simulink model "solar_pv_protected_c07_circuit"  (R2026b)
settings: Solver=VariableStepAuto
model workspace (MAT data in the model file):
  candidate_owner = 'pv_protection_integration_20261023_r01'
  solar_edit_metadata : object (value not decoded)
libraries: fl_lib x149, ee_lib x16, ltc4364demo_lib x3, batteryecm_lib x1, solarprotect_lib x1
(part 11 of 16)

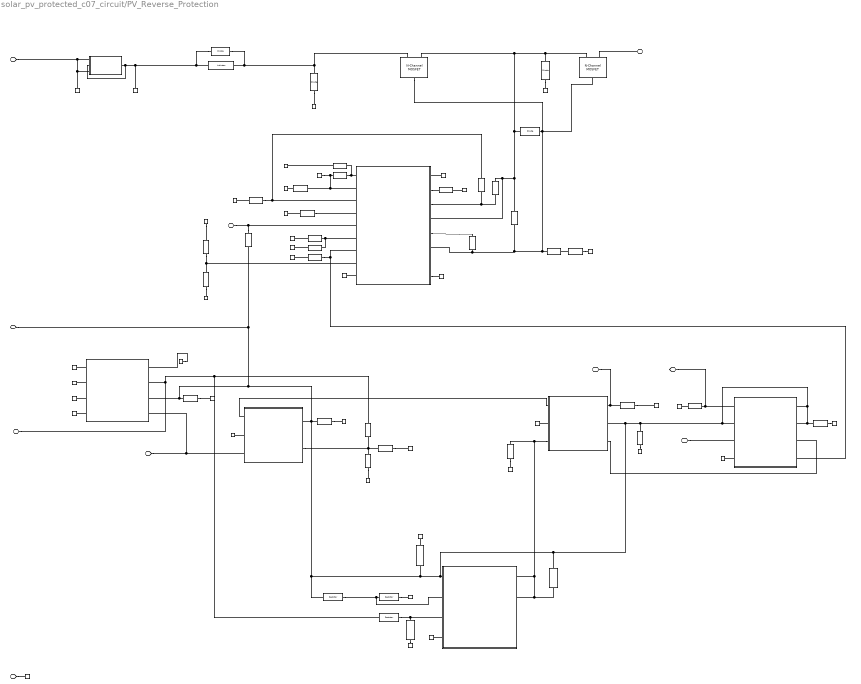
== system solar_pv_protected_c07_circuit/PV_Reverse_Protection ==
  note: L2 / 62 µH / DCR 10 mΩ
  note: PV_C_SUP
      | 100 nF
  note: PV_D_FLY
      | V20PW22-M3/I
  note: PV_D_GS
      | BZT52H-C15,115
  note: PV_D_NEG
      | V20PW22-M3/I
  note: PV_D_TS
      | V20PW22-M3/I
  note: PV_Q1
      | IPB048N15N5LFATMA1
  note: PV_Q2
      | IPB048N15N5LFATMA1
  note: PV_R_SUP25
      | 21.3 kΩ
  note: PV_R_SUP26
      | 10 kΩ
  note: PV_R_SUP31
      | 31.2 kΩ
  note: PV_R_SUP32
      | 10 kΩ
  note: PV_R_SUP_PU
      | 10 kΩ
  note: PV_U6 / TPS37042BJOFDDFRQ1
  note: R27 / 1 mΩ / CSS4J-4026R-1L00F
  note: PV_CBST
      | 10 µF
  note: PV_CTIME
      | 1 nF
  note: PV_CVCC
      | 1 µF
  note: PV_CVIN
      | 100 nF
  note: PV_C_SLEW
      | 100 nF
  note: PV_D_BOOT
      | MMBD1501A
  note: PV_RFLT
      | 100 Ω
  note: PV_RFLT_PU
      | 22 kΩ
  note: PV_RG
      | 100 kΩ
  note: PV_RGS
      | 10 MΩ
  note: PV_RINP
      | 100 kΩ
  note: PV_ROV_H
      | 820 kΩ
  note: PV_ROV_L
      | 10 kΩ
  note: PV_RTIME
      | 100 kΩ
  note: PV_RUV_H
      | 330 kΩ
  note: PV_RUV_L
      | 10.2 kΩ
  note: PV_RVCCUV
      | 113 kΩ
  note: PV_R_SLEW
      | 10 Ω
  note: PV_U1 / LTC7000ARMSE#PBF
  note: C22
      | 100 nF
  note: PV_CREV
      | 10 nF
  note: PV_C_PV_U3
      | 100 nF
  note: PV_RREV_H
      | 10.2 kΩ
  note: PV_RREV_L
      | 9.8 kΩ
  note: PV_U3 / TLV3201AIDBVR
  note: U2 / INA241A3IDDFR
  note: PV_C_PV_U4
      | 100 nF
  note: PV_C_PV_U5
      | 100 nF
  note: PV_RAN
      | 100 kΩ
  note: PV_RREARM
      | 100 kΩ
  note: PV_RRUN
      | 100 kΩ
  note: PV_U4 / SN74LVC1G11DBVR
  note: PV_U5 / SN74LVC1G74DCTR
  note: パネル側の通電・逆流防止回路
  note: R27/U2で電流を検出し、LTC7000Aで保護MOSFET対を開閉する。
      | 逆流判定・停止保持・電源監視によって通電許可を決める。内部はGND以外を直接配線で示す。
  C22 : fl_lib/Electrical/Electrical Elements/Capacitor  Description=|  c=1.0000000000000001e-07 F  r=1e-6 Ohm  g=0 1/Ohm  i_specify=off  i_priority=None  i=0 A  i_nominal_specify=off  i_nominal_value=1  i_nominal_unit=A  v_specify=off  v_priority=None  v=0 V  v_nominal_specify=off  v_nominal_value=1  v_nominal_unit=V  vc_specify=off  vc_priority=High  vc=0 V  vc_nominal_specify=off  vc_nominal_value=1  vc_nominal_unit=V
      | この回路での名前　　; C22
      | 部品名　　　　　　　; C1608X7R1H104K080AA
      | この回路での役割　　; パネル電流を測るU2の3.3 V電源を、瞬間的な変動から支えるためのコンデンサ。
      | ここでの動き　　　　; U2の電源端子と共通GNDの近くで一時的な電流を供給し、速い電流の帰り道を短くする。小さな電流検出信号の配線へ、電源電流の影響を持ち込みにくくする配置を意図する。
      | 
      | 【詳しい働き・仕様・接続・確認の範囲】
      | 部品種別　　　　　　; 積層セラミックコンデンサ（MLCC）
      | 部品分類　　　　　　; 積層セラミックコンデンサ（MLCC）
      | 公称値　　　　　　　; 100nF 50V
      | 配置目的　　　　　　; 電流検出IC電源バイパス。対象ICはU2（INA241A3IDDFR）。
      | 意図する動作　　　　; VS–GNDピン直近。シャントKelvin戻りと電源過渡電流を混ぜない。 各IC局所100nFは同じ3V3でも削減しない。
      | 端子と接続　　　　　; 1 1 → 3V3、2 2 → GND
      | モデルの範囲　　　　; Simscape標準コンデンサの集中定数表現。材質、DCバイアス、周波数依存ESR/ESL、寿命・温度特性を型番から自動再現するモデルではない。
      | モデル設定　　　　　; c=100 nF、r=1 µΩ、g=0 S。これらは保存モデルの設定値であり、すべてが実部品の保証値という意味ではない。
      | 損失の扱い　　　　　; 保存モデルの直列抵抗rと実部品の周波数・温度依存ESRは区別する。容量値が一致しても損失・リプル電流・寿命の成立確認にはならない。
      | 確認の範囲　　　　　; 本説明は保存回路の部品情報・端子割当・既存設計意図を整理したもの。今回の説明更新によって新たな動作試験や実機検証を実施した意味ではない。
      | 設計記録　　　　　　; evaluation\component_annotations_20261022_r01\before_graph.json
      | evaluation\component_annotations_20261022_r01\before_metadata.json
      | evaluation\protection_capacitor_integration_20261021_r01\final_delivery\independent_readback\physical_bom.json
      | evaluation\protection_capacitor_integration_20261021_r01\capacitor_review\capacitor_inventory_after_c04.json
      | evaluation\layout_readability_20261022_r01\capacitor_review\exact_snapshot_capacitor_review.json
      | 
      | 【周波数・ノイズと配置の説明】
      | 周波数面の役割　　　; U2（パネル電流検出IC）の電源端子直近で、瞬間的な電流を供給する局所バイパス。
      | 対象周波数の目安　　; そのICの内部動作や周辺の通信、周囲のスイッチングによる高周波成分を対象にする。100 nFという容量だけから「何MHzまで効く」とは決められない。
      | ノイズの発生源　　　; IC内部の回路動作に伴う電源電流の変化、3.3 V配線を経由する電源変動、近傍のデジタル信号やゲート駆動からの結合。
      | 他のコンデンサとの差; 離れたC18や電源装置側の大きな容量は低い周波数側の蓄積を補う。配線の寄生インダクタンスがあるため、同じ電源ネットでもIC直近の本品を完全に代替できない。
      | 周波数説明の範囲　　; 狙うノイズの周波数と、この部品が実装後に有効な周波数範囲は別である。実効容量、等価直列抵抗、等価直列インダクタンス、配線を含む自己共振で変わるため、型番名や公称容量だけから有効帯域の上限を断定しない。
      | 周波数説明の根拠　　; TDK：Low-ESL Multilayer Ceramic Capacitors
      | https://product.tdk.com/system/files/dam/doc/content/emc-guidebook/en/eemc_product_01.pdf
      | 村田製作所：コンデンサを使いこなす
      | https://www.murata.com/en-GB/products/emc/emifil/library/knowhow/basic/chapter06-p8
      | 
      | 【この説明欄の略語・記号】
      | 用語1　　　　　　　 ; MLCC：Multilayer Ceramic Capacitor（積層セラミックコンデンサ）。薄いセラミック誘電体と電極を重ねたコンデンサ。対象周波数は容量・実装・寄生成分で変わるため、MLCCという分類だけでは決めない。
      | 用語2　　　　　　　 ; ESR：Equivalent Series Resistance（等価直列抵抗）。コンデンサの損失を直列抵抗で表した量。周波数・温度で変わり、損失とリプル電圧に関係する。
      | 用語3　　　　　　　 ; ESL：Equivalent Series Inductance（等価直列インダクタンス）。端子や電極などの寄生インダクタンスを表す。高い周波数ではバイパス効果を制限する。
      | 用語4　　　　　　　 ; DC：Direct Current（直流）。ここでは直流電源または直流成分。DCバイアスはコンデンサに重なる直流電圧を指す。
      | 用語5　　　　　　　 ; IC：Integrated Circuit（集積回路）。複数の電子素子と機能を小さな半導体チップに集積した部品。
      | 用語6　　　　　　　 ; MOSFET：Metal-Oxide-Semiconductor Field-Effect Transistor（金属・酸化膜・半導体構造の電界効果トランジスタ）。ゲートとソースの電圧でドレインとソースの導通を制御する素子。N-MOSはNチャネル型を表す。
      | 用語7　　　　　　　 ; GND：Ground（回路の基準電位・電流帰路）。この図の共通基準。保護接地や大地への接続を意味するとは限らない。
      | 用語8　　　　　　　 ; VCC/VDD/VEE/VS：ICの電源端子名。文字の歴史的な由来を現在の接続機能へ当てはめない。現回路のVEEはU8/U10では浮動基準SW、U9ではGND。各電圧・基準は端子と接続を参照する。
      | 用語9　　　　　　　 ; SW：Switching Node（スイッチング点）。主電力段の上下MOSFETとL1がつながる、電圧が高速に切り替わる点。GNDとは別電位。
      | 
      | 【c06への反映】既存C22をパネル側保護内のU2直近へ移設して再利用。PV_C_U2との二重計上はしない。
  Connection Label{,2,5..7} (5 alike) : ConnectionLabel  Label=panel_pre_shunt
  Connection Label1 : ConnectionLabel  Label=panel_after_shunt
  Connection Label3 : ConnectionLabel  Label=panel_after_shunt
  Connection Label4 : ConnectionLabel  Label=panel_after_shunt
  GND_01 : ConnectionLabel  Description=|  Label=GND
      | 接続名              ; GND
      | 役割                ; この階層の共通基準電位。外部IF_GNDへ接続。
      | 接続端子            ; PV_C_SUP#rconn:1、PV_D_NEG#lconn:1、PV_D_TS#lconn:1、PV_R_SUP26#rconn:1、PV_R_SUP32#rconn:1、PV_U6#lconn:4、IF_GND#rconn:1、PV_CTIME#rconn:1、PV_CVCC#rconn:1、PV_CVIN#rconn:1、PV_C_SLEW#rconn:1、PV_RINP#rconn:1、PV_ROV_L#rconn:1、PV_RTIME#rconn:1、PV_RUV_L#rconn:1、PV_RVCCUV#rconn:1、PV_U1#lconn:9、PV_U1#rconn:8、C22#rconn:1、PV_CREV#rconn:1、PV_C_PV_U3#rconn:1、PV_RREV_L#rconn:1、PV_U3#lconn:2、U2#lconn:2、U2#lconn:3、U2#lconn:4、PV_C_PV_U4#rconn:1、PV_C_PV_U5#rconn:1、PV_RAN#rconn:1、PV_RREARM#rconn:1、PV_RRUN#rconn:1、PV_U4#lconn:2、PV_U5#lconn:4
  GND_02 : ConnectionLabel  Description=|  Label=GND
      | 接続名              ; GND
      | 役割                ; この階層の共通基準電位。外部IF_GNDへ接続。
      | 接続端子            ; PV_C_SUP#rconn:1、PV_D_NEG#lconn:1、PV_D_TS#lconn:1、PV_R_SUP26#rconn:1、PV_R_SUP32#rconn:1、PV_U6#lconn:4、IF_GND#rconn:1、PV_CTIME#rconn:1、PV_CVCC#rconn:1、PV_CVIN#rconn:1、PV_C_SLEW#rconn:1、PV_RINP#rconn:1、PV_ROV_L#rconn:1、PV_RTIME#rconn:1、PV_RUV_L#rconn:1、PV_RVCCUV#rconn:1、PV_U1#lconn:9、PV_U1#rconn:8、C22#rconn:1、PV_CREV#rconn:1、PV_C_PV_U3#rconn:1、PV_RREV_L#rconn:1、PV_U3#lconn:2、U2#lconn:2、U2#lconn:3、U2#lconn:4、PV_C_PV_U4#rconn:1、PV_C_PV_U5#rconn:1、PV_RAN#rconn:1、PV_RREARM#rconn:1、PV_RRUN#rconn:1、PV_U4#lconn:2、PV_U5#lconn:4
  GND_03 : ConnectionLabel  Description=|  Label=GND
      | 接続名              ; GND
      | 役割                ; この階層の共通基準電位。外部IF_GNDへ接続。
      | 接続端子            ; PV_C_SUP#rconn:1、PV_D_NEG#lconn:1、PV_D_TS#lconn:1、PV_R_SUP26#rconn:1、PV_R_SUP32#rconn:1、PV_U6#lconn:4、IF_GND#rconn:1、PV_CTIME#rconn:1、PV_CVCC#rconn:1、PV_CVIN#rconn:1、PV_C_SLEW#rconn:1、PV_RINP#rconn:1、PV_ROV_L#rconn:1、PV_RTIME#rconn:1、PV_RUV_L#rconn:1、PV_RVCCUV#rconn:1、PV_U1#lconn:9、PV_U1#rconn:8、C22#rconn:1、PV_CREV#rconn:1、PV_C_PV_U3#rconn:1、PV_RREV_L#rconn:1、PV_U3#lconn:2、U2#lconn:2、U2#lconn:3、U2#lconn:4、PV_C_PV_U4#rconn:1、PV_C_PV_U5#rconn:1、PV_RAN#rconn:1、PV_RREARM#rconn:1、PV_RRUN#rconn:1、PV_U4#lconn:2、PV_U5#lconn:4
  GND_04 : ConnectionLabel  Description=|  Label=GND
      | 接続名              ; GND
      | 役割                ; この階層の共通基準電位。外部IF_GNDへ接続。
      | 接続端子            ; PV_C_SUP#rconn:1、PV_D_NEG#lconn:1、PV_D_TS#lconn:1、PV_R_SUP26#rconn:1、PV_R_SUP32#rconn:1、PV_U6#lconn:4、IF_GND#rconn:1、PV_CTIME#rconn:1、PV_CVCC#rconn:1、PV_CVIN#rconn:1、PV_C_SLEW#rconn:1、PV_RINP#rconn:1、PV_ROV_L#rconn:1、PV_RTIME#rconn:1、PV_RUV_L#rconn:1、PV_RVCCUV#rconn:1、PV_U1#lconn:9、PV_U1#rconn:8、C22#rconn:1、PV_CREV#rconn:1、PV_C_PV_U3#rconn:1、PV_RREV_L#rconn:1、PV_U3#lconn:2、U2#lconn:2、U2#lconn:3、U2#lconn:4、PV_C_PV_U4#rconn:1、PV_C_PV_U5#rconn:1、PV_RAN#rconn:1、PV_RREARM#rconn:1、PV_RRUN#rconn:1、PV_U4#lconn:2、PV_U5#lconn:4
  GND_05 : ConnectionLabel  Description=|  Label=GND
      | 接続名              ; GND
      | 役割                ; この階層の共通基準電位。外部IF_GNDへ接続。
      | 接続端子            ; PV_C_SUP#rconn:1、PV_D_NEG#lconn:1、PV_D_TS#lconn:1、PV_R_SUP26#rconn:1、PV_R_SUP32#rconn:1、PV_U6#lconn:4、IF_GND#rconn:1、PV_CTIME#rconn:1、PV_CVCC#rconn:1、PV_CVIN#rconn:1、PV_C_SLEW#rconn:1、PV_RINP#rconn:1、PV_ROV_L#rconn:1、PV_RTIME#rconn:1、PV_RUV_L#rconn:1、PV_RVCCUV#rconn:1、PV_U1#lconn:9、PV_U1#rconn:8、C22#rconn:1、PV_CREV#rconn:1、PV_C_PV_U3#rconn:1、PV_RREV_L#rconn:1、PV_U3#lconn:2、U2#lconn:2、U2#lconn:3、U2#lconn:4、PV_C_PV_U4#rconn:1、PV_C_PV_U5#rconn:1、PV_RAN#rconn:1、PV_RREARM#rconn:1、PV_RRUN#rconn:1、PV_U4#lconn:2、PV_U5#lconn:4
  GND_06 : ConnectionLabel  Description=|  Label=GND
      | 接続名              ; GND
      | 役割                ; この階層の共通基準電位。外部IF_GNDへ接続。
      | 接続端子            ; PV_C_SUP#rconn:1、PV_D_NEG#lconn:1、PV_D_TS#lconn:1、PV_R_SUP26#rconn:1、PV_R_SUP32#rconn:1、PV_U6#lconn:4、IF_GND#rconn:1、PV_CTIME#rconn:1、PV_CVCC#rconn:1、PV_CVIN#rconn:1、PV_C_SLEW#rconn:1、PV_RINP#rconn:1、PV_ROV_L#rconn:1、PV_RTIME#rconn:1、PV_RUV_L#rconn:1、PV_RVCCUV#rconn:1、PV_U1#lconn:9、PV_U1#rconn:8、C22#rconn:1、PV_CREV#rconn:1、PV_C_PV_U3#rconn:1、PV_RREV_L#rconn:1、PV_U3#lconn:2、U2#lconn:2、U2#lconn:3、U2#lconn:4、PV_C_PV_U4#rconn:1、PV_C_PV_U5#rconn:1、PV_RAN#rconn:1、PV_RREARM#rconn:1、PV_RRUN#rconn:1、PV_U4#lconn:2、PV_U5#lconn:4
  GND_07 : ConnectionLabel  Description=|  Label=GND
      | 接続名              ; GND
      | 役割                ; この階層の共通基準電位。外部IF_GNDへ接続。
      | 接続端子            ; PV_C_SUP#rconn:1、PV_D_NEG#lconn:1、PV_D_TS#lconn:1、PV_R_SUP26#rconn:1、PV_R_SUP32#rconn:1、PV_U6#lconn:4、IF_GND#rconn:1、PV_CTIME#rconn:1、PV_CVCC#rconn:1、PV_CVIN#rconn:1、PV_C_SLEW#rconn:1、PV_RINP#rconn:1、PV_ROV_L#rconn:1、PV_RTIME#rconn:1、PV_RUV_L#rconn:1、PV_RVCCUV#rconn:1、PV_U1#lconn:9、PV_U1#rconn:8、C22#rconn:1、PV_CREV#rconn:1、PV_C_PV_U3#rconn:1、PV_RREV_L#rconn:1、PV_U3#lconn:2、U2#lconn:2、U2#lconn:3、U2#lconn:4、PV_C_PV_U4#rconn:1、PV_C_PV_U5#rconn:1、PV_RAN#rconn:1、PV_RREARM#rconn:1、PV_RRUN#rconn:1、PV_U4#lconn:2、PV_U5#lconn:4
  GND_08 : ConnectionLabel  Description=|  Label=GND
      | 接続名              ; GND
      | 役割                ; この階層の共通基準電位。外部IF_GNDへ接続。
      | 接続端子            ; PV_C_SUP#rconn:1、PV_D_NEG#lconn:1、PV_D_TS#lconn:1、PV_R_SUP26#rconn:1、PV_R_SUP32#rconn:1、PV_U6#lconn:4、IF_GND#rconn:1、PV_CTIME#rconn:1、PV_CVCC#rconn:1、PV_CVIN#rconn:1、PV_C_SLEW#rconn:1、PV_RINP#rconn:1、PV_ROV_L#rconn:1、PV_RTIME#rconn:1、PV_RUV_L#rconn:1、PV_RVCCUV#rconn:1、PV_U1#lconn:9、PV_U1#rconn:8、C22#rconn:1、PV_CREV#rconn:1、PV_C_PV_U3#rconn:1、PV_RREV_L#rconn:1、PV_U3#lconn:2、U2#lconn:2、U2#lconn:3、U2#lconn:4、PV_C_PV_U4#rconn:1、PV_C_PV_U5#rconn:1、PV_RAN#rconn:1、PV_RREARM#rconn:1、PV_RRUN#rconn:1、PV_U4#lconn:2、PV_U5#lconn:4
  GND_09 : ConnectionLabel  Description=|  Label=GND
      | 接続名              ; GND
      | 役割                ; この階層の共通基準電位。外部IF_GNDへ接続。
      | 接続端子            ; PV_C_SUP#rconn:1、PV_D_NEG#lconn:1、PV_D_TS#lconn:1、PV_R_SUP26#rconn:1、PV_R_SUP32#rconn:1、PV_U6#lconn:4、IF_GND#rconn:1、PV_CTIME#rconn:1、PV_CVCC#rconn:1、PV_CVIN#rconn:1、PV_C_SLEW#rconn:1、PV_RINP#rconn:1、PV_ROV_L#rconn:1、PV_RTIME#rconn:1、PV_RUV_L#rconn:1、PV_RVCCUV#rconn:1、PV_U1#lconn:9、PV_U1#rconn:8、C22#rconn:1、PV_CREV#rconn:1、PV_C_PV_U3#rconn:1、PV_RREV_L#rconn:1、PV_U3#lconn:2、U2#lconn:2、U2#lconn:3、U2#lconn:4、PV_C_PV_U4#rconn:1、PV_C_PV_U5#rconn:1、PV_RAN#rconn:1、PV_RREARM#rconn:1、PV_RRUN#rconn:1、PV_U4#lconn:2、PV_U5#lconn:4
  GND_10 : ConnectionLabel  Description=|  Label=GND
      | 接続名              ; GND
      | 役割                ; この階層の共通基準電位。外部IF_GNDへ接続。
      | 接続端子            ; PV_C_SUP#rconn:1、PV_D_NEG#lconn:1、PV_D_TS#lconn:1、PV_R_SUP26#rconn:1、PV_R_SUP32#rconn:1、PV_U6#lconn:4、IF_GND#rconn:1、PV_CTIME#rconn:1、PV_CVCC#rconn:1、PV_CVIN#rconn:1、PV_C_SLEW#rconn:1、PV_RINP#rconn:1、PV_ROV_L#rconn:1、PV_RTIME#rconn:1、PV_RUV_L#rconn:1、PV_RVCCUV#rconn:1、PV_U1#lconn:9、PV_U1#rconn:8、C22#rconn:1、PV_CREV#rconn:1、PV_C_PV_U3#rconn:1、PV_RREV_L#rconn:1、PV_U3#lconn:2、U2#lconn:2、U2#lconn:3、U2#lconn:4、PV_C_PV_U4#rconn:1、PV_C_PV_U5#rconn:1、PV_RAN#rconn:1、PV_RREARM#rconn:1、PV_RRUN#rconn:1、PV_U4#lconn:2、PV_U5#lconn:4
  GND_11 : ConnectionLabel  Description=|  Label=GND
      | 接続名              ; GND
      | 役割                ; この階層の共通基準電位。外部IF_GNDへ接続。
      | 接続端子            ; PV_C_SUP#rconn:1、PV_D_NEG#lconn:1、PV_D_TS#lconn:1、PV_R_SUP26#rconn:1、PV_R_SUP32#rconn:1、PV_U6#lconn:4、IF_GND#rconn:1、PV_CTIME#rconn:1、PV_CVCC#rconn:1、PV_CVIN#rconn:1、PV_C_SLEW#rconn:1、PV_RINP#rconn:1、PV_ROV_L#rconn:1、PV_RTIME#rconn:1、PV_RUV_L#rconn:1、PV_RVCCUV#rconn:1、PV_U1#lconn:9、PV_U1#rconn:8、C22#rconn:1、PV_CREV#rconn:1、PV_C_PV_U3#rconn:1、PV_RREV_L#rconn:1、PV_U3#lconn:2、U2#lconn:2、U2#lconn:3、U2#lconn:4、PV_C_PV_U4#rconn:1、PV_C_PV_U5#rconn:1、PV_RAN#rconn:1、PV_RREARM#rconn:1、PV_RRUN#rconn:1、PV_U4#lconn:2、PV_U5#lconn:4
  GND_12 : ConnectionLabel  Description=|  Label=GND
      | 接続名              ; GND
      | 役割                ; この階層の共通基準電位。外部IF_GNDへ接続。
      | 接続端子            ; PV_C_SUP#rconn:1、PV_D_NEG#lconn:1、PV_D_TS#lconn:1、PV_R_SUP26#rconn:1、PV_R_SUP32#rconn:1、PV_U6#lconn:4、IF_GND#rconn:1、PV_CTIME#rconn:1、PV_CVCC#rconn:1、PV_CVIN#rconn:1、PV_C_SLEW#rconn:1、PV_RINP#rconn:1、PV_ROV_L#rconn:1、PV_RTIME#rconn:1、PV_RUV_L#rconn:1、PV_RVCCUV#rconn:1、PV_U1#lconn:9、PV_U1#rconn:8、C22#rconn:1、PV_CREV#rconn:1、PV_C_PV_U3#rconn:1、PV_RREV_L#rconn:1、PV_U3#lconn:2、U2#lconn:2、U2#lconn:3、U2#lconn:4、PV_C_PV_U4#rconn:1、PV_C_PV_U5#rconn:1、PV_RAN#rconn:1、PV_RREARM#rconn:1、PV_RRUN#rconn:1、PV_U4#lconn:2、PV_U5#lconn:4
  GND_13 : ConnectionLabel  Description=|  Label=GND
      | 接続名              ; GND
      | 役割                ; この階層の共通基準電位。外部IF_GNDへ接続。
      | 接続端子            ; PV_C_SUP#rconn:1、PV_D_NEG#lconn:1、PV_D_TS#lconn:1、PV_R_SUP26#rconn:1、PV_R_SUP32#rconn:1、PV_U6#lconn:4、IF_GND#rconn:1、PV_CTIME#rconn:1、PV_CVCC#rconn:1、PV_CVIN#rconn:1、PV_C_SLEW#rconn:1、PV_RINP#rconn:1、PV_ROV_L#rconn:1、PV_RTIME#rconn:1、PV_RUV_L#rconn:1、PV_RVCCUV#rconn:1、PV_U1#lconn:9、PV_U1#rconn:8、C22#rconn:1、PV_CREV#rconn:1、PV_C_PV_U3#rconn:1、PV_RREV_L#rconn:1、PV_U3#lconn:2、U2#lconn:2、U2#lconn:3、U2#lconn:4、PV_C_PV_U4#rconn:1、PV_C_PV_U5#rconn:1、PV_RAN#rconn:1、PV_RREARM#rconn:1、PV_RRUN#rconn:1、PV_U4#lconn:2、PV_U5#lconn:4
  GND_14 : ConnectionLabel  Description=|  Label=GND
      | 接続名              ; GND
      | 役割                ; この階層の共通基準電位。外部IF_GNDへ接続。
      | 接続端子            ; PV_C_SUP#rconn:1、PV_D_NEG#lconn:1、PV_D_TS#lconn:1、PV_R_SUP26#rconn:1、PV_R_SUP32#rconn:1、PV_U6#lconn:4、IF_GND#rconn:1、PV_CTIME#rconn:1、PV_CVCC#rconn:1、PV_CVIN#rconn:1、PV_C_SLEW#rconn:1、PV_RINP#rconn:1、PV_ROV_L#rconn:1、PV_RTIME#rconn:1、PV_RUV_L#rconn:1、PV_RVCCUV#rconn:1、PV_U1#lconn:9、PV_U1#rconn:8、C22#rconn:1、PV_CREV#rconn:1、PV_C_PV_U3#rconn:1、PV_RREV_L#rconn:1、PV_U3#lconn:2、U2#lconn:2、U2#lconn:3、U2#lconn:4、PV_C_PV_U4#rconn:1、PV_C_PV_U5#rconn:1、PV_RAN#rconn:1、PV_RREARM#rconn:1、PV_RRUN#rconn:1、PV_U4#lconn:2、PV_U5#lconn:4
  GND_15 : ConnectionLabel  Description=|  Label=GND
      | 接続名              ; GND
      | 役割                ; この階層の共通基準電位。外部IF_GNDへ接続。
      | 接続端子            ; PV_C_SUP#rconn:1、PV_D_NEG#lconn:1、PV_D_TS#lconn:1、PV_R_SUP26#rconn:1、PV_R_SUP32#rconn:1、PV_U6#lconn:4、IF_GND#rconn:1、PV_CTIME#rconn:1、PV_CVCC#rconn:1、PV_CVIN#rconn:1、PV_C_SLEW#rconn:1、PV_RINP#rconn:1、PV_ROV_L#rconn:1、PV_RTIME#rconn:1、PV_RUV_L#rconn:1、PV_RVCCUV#rconn:1、PV_U1#lconn:9、PV_U1#rconn:8、C22#rconn:1、PV_CREV#rconn:1、PV_C_PV_U3#rconn:1、PV_RREV_L#rconn:1、PV_U3#lconn:2、U2#lconn:2、U2#lconn:3、U2#lconn:4、PV_C_PV_U4#rconn:1、PV_C_PV_U5#rconn:1、PV_RAN#rconn:1、PV_RREARM#rconn:1、PV_RRUN#rconn:1、PV_U4#lconn:2、PV_U5#lconn:4
  GND_16 : ConnectionLabel  Description=|  Label=GND
      | 接続名              ; GND
      | 役割                ; この階層の共通基準電位。外部IF_GNDへ接続。
      | 接続端子            ; PV_C_SUP#rconn:1、PV_D_NEG#lconn:1、PV_D_TS#lconn:1、PV_R_SUP26#rconn:1、PV_R_SUP32#rconn:1、PV_U6#lconn:4、IF_GND#rconn:1、PV_CTIME#rconn:1、PV_CVCC#rconn:1、PV_CVIN#rconn:1、PV_C_SLEW#rconn:1、PV_RINP#rconn:1、PV_ROV_L#rconn:1、PV_RTIME#rconn:1、PV_RUV_L#rconn:1、PV_RVCCUV#rconn:1、PV_U1#lconn:9、PV_U1#rconn:8、C22#rconn:1、PV_CREV#rconn:1、PV_C_PV_U3#rconn:1、PV_RREV_L#rconn:1、PV_U3#lconn:2、U2#lconn:2、U2#lconn:3、U2#lconn:4、PV_C_PV_U4#rconn:1、PV_C_PV_U5#rconn:1、PV_RAN#rconn:1、PV_RREARM#rconn:1、PV_RRUN#rconn:1、PV_U4#lconn:2、PV_U5#lconn:4
  GND_17 : ConnectionLabel  Description=|  Label=GND
      | 接続名              ; GND
      | 役割                ; この階層の共通基準電位。外部IF_GNDへ接続。
      | 接続端子            ; PV_C_SUP#rconn:1、PV_D_NEG#lconn:1、PV_D_TS#lconn:1、PV_R_SUP26#rconn:1、PV_R_SUP32#rconn:1、PV_U6#lconn:4、IF_GND#rconn:1、PV_CTIME#rconn:1、PV_CVCC#rconn:1、PV_CVIN#rconn:1、PV_C_SLEW#rconn:1、PV_RINP#rconn:1、PV_ROV_L#rconn:1、PV_RTIME#rconn:1、PV_RUV_L#rconn:1、PV_RVCCUV#rconn:1、PV_U1#lconn:9、PV_U1#rconn:8、C22#rconn:1、PV_CREV#rconn:1、PV_C_PV_U3#rconn:1、PV_RREV_L#rconn:1、PV_U3#lconn:2、U2#lconn:2、U2#lconn:3、U2#lconn:4、PV_C_PV_U4#rconn:1、PV_C_PV_U5#rconn:1、PV_RAN#rconn:1、PV_RREARM#rconn:1、PV_RRUN#rconn:1、PV_U4#lconn:2、PV_U5#lconn:4
  GND_18 : ConnectionLabel  Description=|  Label=GND
      | 接続名              ; GND
      | 役割                ; この階層の共通基準電位。外部IF_GNDへ接続。
      | 接続端子            ; PV_C_SUP#rconn:1、PV_D_NEG#lconn:1、PV_D_TS#lconn:1、PV_R_SUP26#rconn:1、PV_R_SUP32#rconn:1、PV_U6#lconn:4、IF_GND#rconn:1、PV_CTIME#rconn:1、PV_CVCC#rconn:1、PV_CVIN#rconn:1、PV_C_SLEW#rconn:1、PV_RINP#rconn:1、PV_ROV_L#rconn:1、PV_RTIME#rconn:1、PV_RUV_L#rconn:1、PV_RVCCUV#rconn:1、PV_U1#lconn:9、PV_U1#rconn:8、C22#rconn:1、PV_CREV#rconn:1、PV_C_PV_U3#rconn:1、PV_RREV_L#rconn:1、PV_U3#lconn:2、U2#lconn:2、U2#lconn:3、U2#lconn:4、PV_C_PV_U4#rconn:1、PV_C_PV_U5#rconn:1、PV_RAN#rconn:1、PV_RREARM#rconn:1、PV_RRUN#rconn:1、PV_U4#lconn:2、PV_U5#lconn:4
  GND_19 : ConnectionLabel  Description=|  Label=GND
      | 接続名              ; GND
      | 役割                ; この階層の共通基準電位。外部IF_GNDへ接続。
      | 接続端子            ; PV_C_SUP#rconn:1、PV_D_NEG#lconn:1、PV_D_TS#lconn:1、PV_R_SUP26#rconn:1、PV_R_SUP32#rconn:1、PV_U6#lconn:4、IF_GND#rconn:1、PV_CTIME#rconn:1、PV_CVCC#rconn:1、PV_CVIN#rconn:1、PV_C_SLEW#rconn:1、PV_RINP#rconn:1、PV_ROV_L#rconn:1、PV_RTIME#rconn:1、PV_RUV_L#rconn:1、PV_RVCCUV#rconn:1、PV_U1#lconn:9、PV_U1#rconn:8、C22#rconn:1、PV_CREV#rconn:1、PV_C_PV_U3#rconn:1、PV_RREV_L#rconn:1、PV_U3#lconn:2、U2#lconn:2、U2#lconn:3、U2#lconn:4、PV_C_PV_U4#rconn:1、PV_C_PV_U5#rconn:1、PV_RAN#rconn:1、PV_RREARM#rconn:1、PV_RRUN#rconn:1、PV_U4#lconn:2、PV_U5#lconn:4
  GND_20 : ConnectionLabel  Description=|  Label=GND
      | 接続名              ; GND
      | 役割                ; この階層の共通基準電位。外部IF_GNDへ接続。
      | 接続端子            ; PV_C_SUP#rconn:1、PV_D_NEG#lconn:1、PV_D_TS#lconn:1、PV_R_SUP26#rconn:1、PV_R_SUP32#rconn:1、PV_U6#lconn:4、IF_GND#rconn:1、PV_CTIME#rconn:1、PV_CVCC#rconn:1、PV_CVIN#rconn:1、PV_C_SLEW#rconn:1、PV_RINP#rconn:1、PV_ROV_L#rconn:1、PV_RTIME#rconn:1、PV_RUV_L#rconn:1、PV_RVCCUV#rconn:1、PV_U1#lconn:9、PV_U1#rconn:8、C22#rconn:1、PV_CREV#rconn:1、PV_C_PV_U3#rconn:1、PV_RREV_L#rconn:1、PV_U3#lconn:2、U2#lconn:2、U2#lconn:3、U2#lconn:4、PV_C_PV_U4#rconn:1、PV_C_PV_U5#rconn:1、PV_RAN#rconn:1、PV_RREARM#rconn:1、PV_RRUN#rconn:1、PV_U4#lconn:2、PV_U5#lconn:4
  GND_21 : ConnectionLabel  Description=|  Label=GND
      | 接続名              ; GND
      | 役割                ; この階層の共通基準電位。外部IF_GNDへ接続。
      | 接続端子            ; PV_C_SUP#rconn:1、PV_D_NEG#lconn:1、PV_D_TS#lconn:1、PV_R_SUP26#rconn:1、PV_R_SUP32#rconn:1、PV_U6#lconn:4、IF_GND#rconn:1、PV_CTIME#rconn:1、PV_CVCC#rconn:1、PV_CVIN#rconn:1、PV_C_SLEW#rconn:1、PV_RINP#rconn:1、PV_ROV_L#rconn:1、PV_RTIME#rconn:1、PV_RUV_L#rconn:1、PV_RVCCUV#rconn:1、PV_U1#lconn:9、PV_U1#rconn:8、C22#rconn:1、PV_CREV#rconn:1、PV_C_PV_U3#rconn:1、PV_RREV_L#rconn:1、PV_U3#lconn:2、U2#lconn:2、U2#lconn:3、U2#lconn:4、PV_C_PV_U4#rconn:1、PV_C_PV_U5#rconn:1、PV_RAN#rconn:1、PV_RREARM#rconn:1、PV_RRUN#rconn:1、PV_U4#lconn:2、PV_U5#lconn:4
  GND_22 : ConnectionLabel  Description=|  Label=GND
      | 接続名              ; GND
      | 役割                ; この階層の共通基準電位。外部IF_GNDへ接続。
      | 接続端子            ; PV_C_SUP#rconn:1、PV_D_NEG#lconn:1、PV_D_TS#lconn:1、PV_R_SUP26#rconn:1、PV_R_SUP32#rconn:1、PV_U6#lconn:4、IF_GND#rconn:1、PV_CTIME#rconn:1、PV_CVCC#rconn:1、PV_CVIN#rconn:1、PV_C_SLEW#rconn:1、PV_RINP#rconn:1、PV_ROV_L#rconn:1、PV_RTIME#rconn:1、PV_RUV_L#rconn:1、PV_RVCCUV#rconn:1、PV_U1#lconn:9、PV_U1#rconn:8、C22#rconn:1、PV_CREV#rconn:1、PV_C_PV_U3#rconn:1、PV_RREV_L#rconn:1、PV_U3#lconn:2、U2#lconn:2、U2#lconn:3、U2#lconn:4、PV_C_PV_U4#rconn:1、PV_C_PV_U5#rconn:1、PV_RAN#rconn:1、PV_RREARM#rconn:1、PV_RRUN#rconn:1、PV_U4#lconn:2、PV_U5#lconn:4
  GND_23 : ConnectionLabel  Description=|  Label=GND
      | 接続名              ; GND
      | 役割                ; この階層の共通基準電位。外部IF_GNDへ接続。
      | 接続端子            ; PV_C_SUP#rconn:1、PV_D_NEG#lconn:1、PV_D_TS#lconn:1、PV_R_SUP26#rconn:1、PV_R_SUP32#rconn:1、PV_U6#lconn:4、IF_GND#rconn:1、PV_CTIME#rconn:1、PV_CVCC#rconn:1、PV_CVIN#rconn:1、PV_C_SLEW#rconn:1、PV_RINP#rconn:1、PV_ROV_L#rconn:1、PV_RTIME#rconn:1、PV_RUV_L#rconn:1、PV_RVCCUV#rconn:1、PV_U1#lconn:9、PV_U1#rconn:8、C22#rconn:1、PV_CREV#rconn:1、PV_C_PV_U3#rconn:1、PV_RREV_L#rconn:1、PV_U3#lconn:2、U2#lconn:2、U2#lconn:3、U2#lconn:4、PV_C_PV_U4#rconn:1、PV_C_PV_U5#rconn:1、PV_RAN#rconn:1、PV_RREARM#rconn:1、PV_RRUN#rconn:1、PV_U4#lconn:2、PV_U5#lconn:4
  GND_24 : ConnectionLabel  Description=|  Label=GND
      | 接続名              ; GND
      | 役割                ; この階層の共通基準電位。外部IF_GNDへ接続。
      | 接続端子            ; PV_C_SUP#rconn:1、PV_D_NEG#lconn:1、PV_D_TS#lconn:1、PV_R_SUP26#rconn:1、PV_R_SUP32#rconn:1、PV_U6#lconn:4、IF_GND#rconn:1、PV_CTIME#rconn:1、PV_CVCC#rconn:1、PV_CVIN#rconn:1、PV_C_SLEW#rconn:1、PV_RINP#rconn:1、PV_ROV_L#rconn:1、PV_RTIME#rconn:1、PV_RUV_L#rconn:1、PV_RVCCUV#rconn:1、PV_U1#lconn:9、PV_U1#rconn:8、C22#rconn:1、PV_CREV#rconn:1、PV_C_PV_U3#rconn:1、PV_RREV_L#rconn:1、PV_U3#lconn:2、U2#lconn:2、U2#lconn:3、U2#lconn:4、PV_C_PV_U4#rconn:1、PV_C_PV_U5#rconn:1、PV_RAN#rconn:1、PV_RREARM#rconn:1、PV_RRUN#rconn:1、PV_U4#lconn:2、PV_U5#lconn:4
  GND_25 : ConnectionLabel  Description=|  Label=GND
      | 接続名              ; GND
      | 役割                ; この階層の共通基準電位。外部IF_GNDへ接続。
      | 接続端子            ; PV_C_SUP#rconn:1、PV_D_NEG#lconn:1、PV_D_TS#lconn:1、PV_R_SUP26#rconn:1、PV_R_SUP32#rconn:1、PV_U6#lconn:4、IF_GND#rconn:1、PV_CTIME#rconn:1、PV_CVCC#rconn:1、PV_CVIN#rconn:1、PV_C_SLEW#rconn:1、PV_RINP#rconn:1、PV_ROV_L#rconn:1、PV_RTIME#rconn:1、PV_RUV_L#rconn:1、PV_RVCCUV#rconn:1、PV_U1#lconn:9、PV_U1#rconn:8、C22#rconn:1、PV_CREV#rconn:1、PV_C_PV_U3#rconn:1、PV_RREV_L#rconn:1、PV_U3#lconn:2、U2#lconn:2、U2#lconn:3、U2#lconn:4、PV_C_PV_U4#rconn:1、PV_C_PV_U5#rconn:1、PV_RAN#rconn:1、PV_RREARM#rconn:1、PV_RRUN#rconn:1、PV_U4#lconn:2、PV_U5#lconn:4
  GND_26 : ConnectionLabel  Description=|  Label=GND
      | 接続名              ; GND
      | 役割                ; この階層の共通基準電位。外部IF_GNDへ接続。
      | 接続端子            ; PV_C_SUP#rconn:1、PV_D_NEG#lconn:1、PV_D_TS#lconn:1、PV_R_SUP26#rconn:1、PV_R_SUP32#rconn:1、PV_U6#lconn:4、IF_GND#rconn:1、PV_CTIME#rconn:1、PV_CVCC#rconn:1、PV_CVIN#rconn:1、PV_C_SLEW#rconn:1、PV_RINP#rconn:1、PV_ROV_L#rconn:1、PV_RTIME#rconn:1、PV_RUV_L#rconn:1、PV_RVCCUV#rconn:1、PV_U1#lconn:9、PV_U1#rconn:8、C22#rconn:1、PV_CREV#rconn:1、PV_C_PV_U3#rconn:1、PV_RREV_L#rconn:1、PV_U3#lconn:2、U2#lconn:2、U2#lconn:3、U2#lconn:4、PV_C_PV_U4#rconn:1、PV_C_PV_U5#rconn:1、PV_RAN#rconn:1、PV_RREARM#rconn:1、PV_RRUN#rconn:1、PV_U4#lconn:2、PV_U5#lconn:4
  GND_27 : ConnectionLabel  Description=|  Label=GND
      | 接続名              ; GND
      | 役割                ; この階層の共通基準電位。外部IF_GNDへ接続。
      | 接続端子            ; PV_C_SUP#rconn:1、PV_D_NEG#lconn:1、PV_D_TS#lconn:1、PV_R_SUP26#rconn:1、PV_R_SUP32#rconn:1、PV_U6#lconn:4、IF_GND#rconn:1、PV_CTIME#rconn:1、PV_CVCC#rconn:1、PV_CVIN#rconn:1、PV_C_SLEW#rconn:1、PV_RINP#rconn:1、PV_ROV_L#rconn:1、PV_RTIME#rconn:1、PV_RUV_L#rconn:1、PV_RVCCUV#rconn:1、PV_U1#lconn:9、PV_U1#rconn:8、C22#rconn:1、PV_CREV#rconn:1、PV_C_PV_U3#rconn:1、PV_RREV_L#rconn:1、PV_U3#lconn:2、U2#lconn:2、U2#lconn:3、U2#lconn:4、PV_C_PV_U4#rconn:1、PV_C_PV_U5#rconn:1、PV_RAN#rconn:1、PV_RREARM#rconn:1、PV_RRUN#rconn:1、PV_U4#lconn:2、PV_U5#lconn:4
  GND_28 : ConnectionLabel  Description=|  Label=GND
      | 接続名              ; GND
      | 役割                ; この階層の共通基準電位。外部IF_GNDへ接続。
      | 接続端子            ; PV_C_SUP#rconn:1、PV_D_NEG#lconn:1、PV_D_TS#lconn:1、PV_R_SUP26#rconn:1、PV_R_SUP32#rconn:1、PV_U6#lconn:4、IF_GND#rconn:1、PV_CTIME#rconn:1、PV_CVCC#rconn:1、PV_CVIN#rconn:1、PV_C_SLEW#rconn:1、PV_RINP#rconn:1、PV_ROV_L#rconn:1、PV_RTIME#rconn:1、PV_RUV_L#rconn:1、PV_RVCCUV#rconn:1、PV_U1#lconn:9、PV_U1#rconn:8、C22#rconn:1、PV_CREV#rconn:1、PV_C_PV_U3#rconn:1、PV_RREV_L#rconn:1、PV_U3#lconn:2、U2#lconn:2、U2#lconn:3、U2#lconn:4、PV_C_PV_U4#rconn:1、PV_C_PV_U5#rconn:1、PV_RAN#rconn:1、PV_RREARM#rconn:1、PV_RRUN#rconn:1、PV_U4#lconn:2、PV_U5#lconn:4
  GND_29 : ConnectionLabel  Description=|  Label=GND
      | 接続名              ; GND
      | 役割                ; この階層の共通基準電位。外部IF_GNDへ接続。
      | 接続端子            ; PV_C_SUP#rconn:1、PV_D_NEG#lconn:1、PV_D_TS#lconn:1、PV_R_SUP26#rconn:1、PV_R_SUP32#rconn:1、PV_U6#lconn:4、IF_GND#rconn:1、PV_CTIME#rconn:1、PV_CVCC#rconn:1、PV_CVIN#rconn:1、PV_C_SLEW#rconn:1、PV_RINP#rconn:1、PV_ROV_L#rconn:1、PV_RTIME#rconn:1、PV_RUV_L#rconn:1、PV_RVCCUV#rconn:1、PV_U1#lconn:9、PV_U1#rconn:8、C22#rconn:1、PV_CREV#rconn:1、PV_C_PV_U3#rconn:1、PV_RREV_L#rconn:1、PV_U3#lconn:2、U2#lconn:2、U2#lconn:3、U2#lconn:4、PV_C_PV_U4#rconn:1、PV_C_PV_U5#rconn:1、PV_RAN#rconn:1、PV_RREARM#rconn:1、PV_RRUN#rconn:1、PV_U4#lconn:2、PV_U5#lconn:4
  GND_30 : ConnectionLabel  Description=|  Label=GND
      | 接続名              ; GND
      | 役割                ; この階層の共通基準電位。外部IF_GNDへ接続。
      | 接続端子            ; PV_C_SUP#rconn:1、PV_D_NEG#lconn:1、PV_D_TS#lconn:1、PV_R_SUP26#rconn:1、PV_R_SUP32#rconn:1、PV_U6#lconn:4、IF_GND#rconn:1、PV_CTIME#rconn:1、PV_CVCC#rconn:1、PV_CVIN#rconn:1、PV_C_SLEW#rconn:1、PV_RINP#rconn:1、PV_ROV_L#rconn:1、PV_RTIME#rconn:1、PV_RUV_L#rconn:1、PV_RVCCUV#rconn:1、PV_U1#lconn:9、PV_U1#rconn:8、C22#rconn:1、PV_CREV#rconn:1、PV_C_PV_U3#rconn:1、PV_RREV_L#rconn:1、PV_U3#lconn:2、U2#lconn:2、U2#lconn:3、U2#lconn:4、PV_C_PV_U4#rconn:1、PV_C_PV_U5#rconn:1、PV_RAN#rconn:1、PV_RREARM#rconn:1、PV_RRUN#rconn:1、PV_U4#lconn:2、PV_U5#lconn:4
  GND_31 : ConnectionLabel  Description=|  Label=GND
      | 接続名              ; GND
      | 役割                ; この階層の共通基準電位。外部IF_GNDへ接続。
      | 接続端子            ; PV_C_SUP#rconn:1、PV_D_NEG#lconn:1、PV_D_TS#lconn:1、PV_R_SUP26#rconn:1、PV_R_SUP32#rconn:1、PV_U6#lconn:4、IF_GND#rconn:1、PV_CTIME#rconn:1、PV_CVCC#rconn:1、PV_CVIN#rconn:1、PV_C_SLEW#rconn:1、PV_RINP#rconn:1、PV_ROV_L#rconn:1、PV_RTIME#rconn:1、PV_RUV_L#rconn:1、PV_RVCCUV#rconn:1、PV_U1#lconn:9、PV_U1#rconn:8、C22#rconn:1、PV_CREV#rconn:1、PV_C_PV_U3#rconn:1、PV_RREV_L#rconn:1、PV_U3#lconn:2、U2#lconn:2、U2#lconn:3、U2#lconn:4、PV_C_PV_U4#rconn:1、PV_C_PV_U5#rconn:1、PV_RAN#rconn:1、PV_RREARM#rconn:1、PV_RRUN#rconn:1、PV_U4#lconn:2、PV_U5#lconn:4
  GND_32 : ConnectionLabel  Description=|  Label=GND
      | 接続名              ; GND
      | 役割                ; この階層の共通基準電位。外部IF_GNDへ接続。
      | 接続端子            ; PV_C_SUP#rconn:1、PV_D_NEG#lconn:1、PV_D_TS#lconn:1、PV_R_SUP26#rconn:1、PV_R_SUP32#rconn:1、PV_U6#lconn:4、IF_GND#rconn:1、PV_CTIME#rconn:1、PV_CVCC#rconn:1、PV_CVIN#rconn:1、PV_C_SLEW#rconn:1、PV_RINP#rconn:1、PV_ROV_L#rconn:1、PV_RTIME#rconn:1、PV_RUV_L#rconn:1、PV_RVCCUV#rconn:1、PV_U1#lconn:9、PV_U1#rconn:8、C22#rconn:1、PV_CREV#rconn:1、PV_C_PV_U3#rconn:1、PV_RREV_L#rconn:1、PV_U3#lconn:2、U2#lconn:2、U2#lconn:3、U2#lconn:4、PV_C_PV_U4#rconn:1、PV_C_PV_U5#rconn:1、PV_RAN#rconn:1、PV_RREARM#rconn:1、PV_RRUN#rconn:1、PV_U4#lconn:2、PV_U5#lconn:4
  GND_33 : ConnectionLabel  Description=|  Label=GND
      | 接続名              ; GND
      | 役割                ; この階層の共通基準電位。外部IF_GNDへ接続。
      | 接続端子            ; PV_C_SUP#rconn:1、PV_D_NEG#lconn:1、PV_D_TS#lconn:1、PV_R_SUP26#rconn:1、PV_R_SUP32#rconn:1、PV_U6#lconn:4、IF_GND#rconn:1、PV_CTIME#rconn:1、PV_CVCC#rconn:1、PV_CVIN#rconn:1、PV_C_SLEW#rconn:1、PV_RINP#rconn:1、PV_ROV_L#rconn:1、PV_RTIME#rconn:1、PV_RUV_L#rconn:1、PV_RVCCUV#rconn:1、PV_U1#lconn:9、PV_U1#rconn:8、C22#rconn:1、PV_CREV#rconn:1、PV_C_PV_U3#rconn:1、PV_RREV_L#rconn:1、PV_U3#lconn:2、U2#lconn:2、U2#lconn:3、U2#lconn:4、PV_C_PV_U4#rconn:1、PV_C_PV_U5#rconn:1、PV_RAN#rconn:1、PV_RREARM#rconn:1、PV_RRUN#rconn:1、PV_U4#lconn:2、PV_U5#lconn:4
  L2 : fl_lib/Electrical/Electrical Elements/Inductor  Description=|  l=62e-6 H  r=0.01 Ohm  g=1e-9 1/Ohm  i_specify=off  i_priority=None  i=0 A  i_nominal_specify=off  i_nominal_value=1  i_nominal_unit=A  v_specify=off  v_priority=None  v=0 V  v_nominal_specify=off  v_nominal_value=1  v_nominal_unit=V  i_L_specify=off  i_L_priority=High  i_L=0 A  i_L_nominal_specify=off  i_L_nominal_value=1  i_L_nominal_unit=A
      | この回路での名前    ; L2
      | 部品名              ; 74437636356203
      | この回路での役割    ; 主電力段が入力側へ返すスイッチング電流の変動を和らげる62 µHの入力フィルタ用インダクタ。
      | ここでの動き        ; 既存L2をシャントR27より後、保護MOSFET対より前へ移す。保護が開く瞬間の蓄積エネルギーを周辺クランプへ逃がす構成と一緒に評価する。
      | 保存モデル値        ; L=62e-6 H、直列抵抗=0.01 Ω。これらは実行モデルに保存された値で、実部品の全温度・全電流特性を保証する値とは限らない。
      | モデルの範囲        ; Simscape標準インダクタ。飽和・温度・巻線寄生と実部品の保証範囲は別評価。
      | 用語                ; µH：マイクロヘンリー。MOSFET：Metal-Oxide-Semiconductor Field-Effect Transistor（金属・酸化膜・半導体構造の電界効果トランジスタ）。
  PV_CBST : fl_lib/Electrical/Electrical Elements/Capacitor  Description=|  c=10e-6 F  r=1e-6 Ohm  g=0 1/Ohm  i_specify=off  i_priority=None  i=0 A  i_nominal_specify=off  i_nominal_value=1  i_nominal_unit=A  v_specify=off  v_priority=None  v=0 V  v_nominal_specify=off  v_nominal_value=1  v_nominal_unit=V  vc_specify=on  vc_priority=High  vc=0 V  vc_nominal_specify=off  vc_nominal_value=1  vc_nominal_unit=V
      | この回路での名前    ; PV_CBST
      | 部品名              ; 型番未選定 / 保存定数を使用
      | この回路での役割    ; LTC7000AがMOSFETのゲートを充電するための浮動電源の蓄電コンデンサ。BSTと共通ソースTSの間に置く。25V級を候補とし、実効容量と充電時間を確認する。
      | 保存モデル値        ; c=10e-6
      | この図の範囲        ; この図面は実部品の端子と接続を示す。保存実行モジュール SHA256=f40bf5e1ef20bc97d0d4775a6ac457f3c30378c5fe9d07d29ab7bde4d975da32 の数値計算用ICコアを図面コピーから除去してある。実行用のICはメーカーのトランジスタモデルではなく、限定範囲の近似動作モデル。試験の合否と条件は C:\Users\hosik\OneDrive\ドキュメント\ChatGPT\oosem\evaluation\pv_protection_integration_20261023_r01\runtime\observations\standard_final_r04_aggregate\aggregate.json を参照する。
      | 注意                ; ゲート漏れ・チャージポンプの電流・起動時の電荷量・部品公差に依存する。値だけで突入や起動を保証しない。
  PV_CREV : fl_lib/Electrical/Electrical Elements/Capacitor  Description=|  c=1e-08 F  r=1e-6 Ohm  g=0 1/Ohm  i_specify=off  i_priority=None  i=0 A  i_nominal_specify=off  i_nominal_value=1  i_nominal_unit=A  v_specify=off  v_priority=None  v=0 V  v_nominal_specify=off  v_nominal_value=1  v_nominal_unit=V  vc_specify=off  vc_priority=High  vc=0 V  vc_nominal_specify=off  vc_nominal_value=1  vc_nominal_unit=V
      | この回路での名前    ; PV_CREV
      | 部品名              ; 未選定 / 10 nF / 16 V
      | この回路での役割    ; 判定用基準電圧の局所ノイズを抑える。立上り待ち時間に含める。
      | ここでの動き        ; V_REV と GND の間に配置。支援するIC近傍へ置く。
      | 公称値              ; 10 nF / 16 V
      | 採用状態            ; 図面化のための候補定数。動作・SOA・熱・ノイズの成立から再調整する。
      | モデルの範囲        ; Simscape標準Capacitor。型番の周波数依存・温度依存特性を同定したモデルではない。
      | 用語と選定の注意    ; MLCC：Multilayer Ceramic Capacitor（積層セラミックコンデンサ）を候補とする。ICの切替えやゲート充放電が生む局所的な高周波電流を支える。容量だけで周波数特性は決まらず、実効容量・ESR・ESLと配置の確認が必要。DC：Direct Current（直流）。ESR：Equivalent Series Resistance（等価直列抵抗）。ESL：Equivalent Series Inductance（等価直列インダクタンス）。
  PV_CTIME : fl_lib/Electrical/Electrical Elements/Capacitor  Description=|  c=1.0000000000000001e-09 F  r=1e-6 Ohm  g=0 1/Ohm  i_specify=off  i_priority=None  i=0 A  i_nominal_specify=off  i_nominal_value=1  i_nominal_unit=A  v_specify=off  v_priority=None  v=0 V  v_nominal_specify=off  v_nominal_value=1  v_nominal_unit=V  vc_specify=off  vc_priority=High  vc=0 V  vc_nominal_specify=off  vc_nominal_value=1  vc_nominal_unit=V
      | この回路での名前    ; PV_CTIME
      | 部品名              ; 未選定 / 1 nF / 25 V
      | この回路での役割    ; 過電流遮断遅延の仮値。100k並列の影響も含めSOAと突入から要調整。
      | ここでの動き        ; PV_TIMER と GND の間に配置。支援するIC近傍へ置く。
      | 公称値              ; 1 nF / 25 V
      | 採用状態            ; 図面化のための候補定数。動作・SOA・熱・ノイズの成立から再調整する。
      | モデルの範囲        ; Simscape標準Capacitor。型番の周波数依存・温度依存特性を同定したモデルではない。
      | 用語と選定の注意    ; MLCC：Multilayer Ceramic Capacitor（積層セラミックコンデンサ）を候補とする。ICの切替えやゲート充放電が生む局所的な高周波電流を支える。容量だけで周波数特性は決まらず、実効容量・ESR・ESLと配置の確認が必要。DC：Direct Current（直流）。ESR：Equivalent Series Resistance（等価直列抵抗）。ESL：Equivalent Series Inductance（等価直列インダクタンス）。
  PV_CVCC : fl_lib/Electrical/Electrical Elements/Capacitor  Description=|  c=9.9999999999999995e-07 F  r=1e-6 Ohm  g=0 1/Ohm  i_specify=off  i_priority=None  i=0 A  i_nominal_specify=off  i_nominal_value=1  i_nominal_unit=A  v_specify=off  v_priority=None  v=0 V  v_nominal_specify=off  v_nominal_value=1  v_nominal_unit=V  vc_specify=off  vc_priority=High  vc=0 V  vc_nominal_specify=off  vc_nominal_value=1  vc_nominal_unit=V
      | この回路での名前    ; PV_CVCC
      | 部品名              ; 未選定 / 1 uF / 25 V
      | この回路での役割    ; 内部10V電源の局所バイパス。DCバイアス後の実効容量も確認する。
      | ここでの動き        ; PV_DRV_VCC と GND の間に配置。支援するIC近傍へ置く。
      | 公称値              ; 1 uF / 25 V
      | 採用状態            ; 図面化のための候補定数。動作・SOA・熱・ノイズの成立から再調整する。
      | モデルの範囲        ; Simscape標準Capacitor。型番の周波数依存・温度依存特性を同定したモデルではない。
      | 用語と選定の注意    ; MLCC：Multilayer Ceramic Capacitor（積層セラミックコンデンサ）を候補とする。ICの切替えやゲート充放電が生む局所的な高周波電流を支える。容量だけで周波数特性は決まらず、実効容量・ESR・ESLと配置の確認が必要。DC：Direct Current（直流）。ESR：Equivalent Series Resistance（等価直列抵抗）。ESL：Equivalent Series Inductance（等価直列インダクタンス）。
  PV_CVIN : fl_lib/Electrical/Electrical Elements/Capacitor  Description=|  c=1.0000000000000001e-07 F  r=1e-6 Ohm  g=0 1/Ohm  i_specify=off  i_priority=None  i=0 A  i_nominal_specify=off  i_nominal_value=1  i_nominal_unit=A  v_specify=off  v_priority=None  v=0 V  v_nominal_specify=off  v_nominal_value=1  v_nominal_unit=V  vc_specify=off  vc_priority=High  vc=0 V  vc_nominal_specify=off  vc_nominal_value=1  vc_nominal_unit=V
      | この回路での名前    ; PV_CVIN
      | 部品名              ; 未選定 / 100 nF / 200 V
      | この回路での役割    ; 保護ICの高電圧入力電源を局所的に安定化する。
      | ここでの動き        ; PV_IN と GND の間に配置。支援するIC近傍へ置く。
      | 公称値              ; 100 nF / 200 V
      | 採用状態            ; 図面化のための候補定数。動作・SOA・熱・ノイズの成立から再調整する。
      | モデルの範囲        ; Simscape標準Capacitor。型番の周波数依存・温度依存特性を同定したモデルではない。
      | 用語と選定の注意    ; MLCC：Multilayer Ceramic Capacitor（積層セラミックコンデンサ）を候補とする。ICの切替えやゲート充放電が生む局所的な高周波電流を支える。容量だけで周波数特性は決まらず、実効容量・ESR・ESLと配置の確認が必要。DC：Direct Current（直流）。ESR：Equivalent Series Resistance（等価直列抵抗）。ESL：Equivalent Series Inductance（等価直列インダクタンス）。
  PV_C_PV_U3 : fl_lib/Electrical/Electrical Elements/Capacitor  Description=|  c=1.0000000000000001e-07 F  r=1e-6 Ohm  g=0 1/Ohm  i_specify=off  i_priority=None  i=0 A  i_nominal_specify=off  i_nominal_value=1  i_nominal_unit=A  v_specify=off  v_priority=None  v=0 V  v_nominal_specify=off  v_nominal_value=1  v_nominal_unit=V  vc_specify=off  vc_priority=High  vc=0 V  vc_nominal_specify=off  vc_nominal_value=1  vc_nominal_unit=V
      | この回路での名前    ; PV_C_PV_U3
      | 部品名              ; 未選定 / 100 nF / 16 V
      | この回路での役割    ; PV_U3の電源ピンのすぐ近くに置くデカップリング。
      | ここでの動き        ; P3V3 と GND の間に配置。支援するIC近傍へ置く。
      | 公称値              ; 100 nF / 16 V
      | 採用状態            ; 図面化のための候補定数。動作・SOA・熱・ノイズの成立から再調整する。
      | モデルの範囲        ; Simscape標準Capacitor。型番の周波数依存・温度依存特性を同定したモデルではない。
      | 用語と選定の注意    ; MLCC：Multilayer Ceramic Capacitor（積層セラミックコンデンサ）を候補とする。ICの切替えやゲート充放電が生む局所的な高周波電流を支える。容量だけで周波数特性は決まらず、実効容量・ESR・ESLと配置の確認が必要。DC：Direct Current（直流）。ESR：Equivalent Series Resistance（等価直列抵抗）。ESL：Equivalent Series Inductance（等価直列インダクタンス）。
  PV_C_PV_U4 : fl_lib/Electrical/Electrical Elements/Capacitor  Description=|  c=1.0000000000000001e-07 F  r=1e-6 Ohm  g=0 1/Ohm  i_specify=off  i_priority=None  i=0 A  i_nominal_specify=off  i_nominal_value=1  i_nominal_unit=A  v_specify=off  v_priority=None  v=0 V  v_nominal_specify=off  v_nominal_value=1  v_nominal_unit=V  vc_specify=off  vc_priority=High  vc=0 V  vc_nominal_specify=off  vc_nominal_value=1  vc_nominal_unit=V
      | この回路での名前    ; PV_C_PV_U4
      | 部品名              ; 未選定 / 100 nF / 16 V
      | この回路での役割    ; PV_U4の電源ピンのすぐ近くに置くデカップリング。
      | ここでの動き        ; P3V3 と GND の間に配置。支援するIC近傍へ置く。
      | 公称値              ; 100 nF / 16 V
      | 採用状態            ; 図面化のための候補定数。動作・SOA・熱・ノイズの成立から再調整する。
      | モデルの範囲        ; Simscape標準Capacitor。型番の周波数依存・温度依存特性を同定したモデルではない。
      | 用語と選定の注意    ; MLCC：Multilayer Ceramic Capacitor（積層セラミックコンデンサ）を候補とする。ICの切替えやゲート充放電が生む局所的な高周波電流を支える。容量だけで周波数特性は決まらず、実効容量・ESR・ESLと配置の確認が必要。DC：Direct Current（直流）。ESR：Equivalent Series Resistance（等価直列抵抗）。ESL：Equivalent Series Inductance（等価直列インダクタンス）。
  PV_C_PV_U5 : fl_lib/Electrical/Electrical Elements/Capacitor  Description=|  c=1.0000000000000001e-07 F  r=1e-6 Ohm  g=0 1/Ohm  i_specify=off  i_priority=None  i=0 A  i_nominal_specify=off  i_nominal_value=1  i_nominal_unit=A  v_specify=off  v_priority=None  v=0 V  v_nominal_specify=off  v_nominal_value=1  v_nominal_unit=V  vc_specify=off  vc_priority=High  vc=0 V  vc_nominal_specify=off  vc_nominal_value=1  vc_nominal_unit=V
      | この回路での名前    ; PV_C_PV_U5
      | 部品名              ; 未選定 / 100 nF / 16 V
      | この回路での役割    ; PV_U5の電源ピンのすぐ近くに置くデカップリング。
      | ここでの動き        ; P3V3 と GND の間に配置。支援するIC近傍へ置く。
      | 公称値              ; 100 nF / 16 V
      | 採用状態            ; 図面化のための候補定数。動作・SOA・熱・ノイズの成立から再調整する。
      | モデルの範囲        ; Simscape標準Capacitor。型番の周波数依存・温度依存特性を同定したモデルではない。
      | 用語と選定の注意    ; MLCC：Multilayer Ceramic Capacitor（積層セラミックコンデンサ）を候補とする。ICの切替えやゲート充放電が生む局所的な高周波電流を支える。容量だけで周波数特性は決まらず、実効容量・ESR・ESLと配置の確認が必要。DC：Direct Current（直流）。ESR：Equivalent Series Resistance（等価直列抵抗）。ESL：Equivalent Series Inductance（等価直列インダクタンス）。
  PV_C_SLEW : fl_lib/Electrical/Electrical Elements/Capacitor  Description=|  c=100e-9 F  r=1e-6 Ohm  g=0 1/Ohm  i_specify=off  i_priority=None  i=0 A  i_nominal_specify=off  i_nominal_value=1  i_nominal_unit=A  v_specify=off  v_priority=None  v=0 V  v_nominal_specify=off  v_nominal_value=1  v_nominal_unit=V  vc_specify=on  vc_priority=High  vc=0 V  vc_nominal_specify=off  vc_nominal_value=1  vc_nominal_unit=V
      | この回路での名前    ; PV_C_SLEW
      | 部品名              ; 型番未選定 / 100 nF / 200 V
      | この回路での役割    ; 保護MOSFETをONするときのゲート上昇を遅くし、入力コンデンサへの突入電流を抑えるための追加容量。
      | ここでの動き        ; 100nF、200V級を選定する。ゲートと共通ソース間ではなくGNDへ接続するので、PV電圧に駆動分が重なった電圧を受ける。DCバイアス下の実効容量を確認する。
      | 端子と接続          ; PV_SLEW と GND の間
      | 保存モデル値        ; c=100e-9
      | 選定の範囲          ; 保存モデルの定数を表す。実部品の型番・公差・電力・温度・周波数依存の最終選定は別。ここではモデルの値や接続を変更していない。
      | メーカー根拠        ; LTC7000A Fig.12: https://www.analog.com/media/en/technical-documentation/data-sheets/ltc7000a.pdf 。TPS3704: https://www.ti.com/lit/ds/symlink/tps3704.pdf
      | 用語                ; MLCC：Multilayer Ceramic Capacitor（積層セラミックコンデンサ）。DC：Direct Current（直流）。バイパス容量はICの切替時に生じる高周波電流の局所帰路を作る。狙う周波数は容量だけでなく実効容量・ESR（等価直列抵抗）・ESL（等価直列インダクタンス）と配置で決まる。
  PV_C_SUP : fl_lib/Electrical/Electrical Elements/Capacitor  Description=|  c=100e-9 F  r=1e-6 Ohm  g=0 1/Ohm  i_specify=off  i_priority=None  i=0 A  i_nominal_specify=off  i_nominal_value=1  i_nominal_unit=A  v_specify=off  v_priority=None  v=0 V  v_nominal_specify=off  v_nominal_value=1  v_nominal_unit=V  vc_specify=on  vc_priority=High  vc=0 V  vc_nominal_specify=off  vc_nominal_value=1  vc_nominal_unit=V
      | この回路での名前    ; PV_C_SUP
      | 部品名              ; 型番未選定 / 100 nF
      | この回路での役割    ; PV_U6の電源を局所的に安定させるバイパスコンデンサ。
      | ここでの動き        ; 100nFをPV_U6のVDD/GNDのすぐ近くへ置き、電源ループを短くする。
      | 端子と接続          ; P3V3 と GND の間
      | 保存モデル値        ; c=100e-9
      | 選定の範囲          ; 保存モデルの定数を表す。実部品の型番・公差・電力・温度・周波数依存の最終選定は別。ここではモデルの値や接続を変更していない。
      | メーカー根拠        ; LTC7000A Fig.12: https://www.analog.com/media/en/technical-documentation/data-sheets/ltc7000a.pdf 。TPS3704: https://www.ti.com/lit/ds/symlink/tps3704.pdf
      | 用語                ; MLCC：Multilayer Ceramic Capacitor（積層セラミックコンデンサ）。DC：Direct Current（直流）。バイパス容量はICの切替時に生じる高周波電流の局所帰路を作る。狙う周波数は容量だけでなく実効容量・ESR（等価直列抵抗）・ESL（等価直列インダクタンス）と配置で決まる。
  PV_D_BOOT : fl_lib/Electrical/Electrical Elements/Diode  Description=|  Vf=0.8 V  Ron=5 Ohm  Goff=1e-8 1/Ohm  i_specify=off  i_priority=None  i=0 A  i_nominal_specify=off  i_nominal_value=1  i_nominal_unit=A  v_specify=off  v_priority=None  v=0 V  v_nominal_specify=off  v_nominal_value=1  v_nominal_unit=V
      | この回路での名前    ; PV_D_BOOT
      | 部品名              ; onsemi MMBD1501A（候補）
      | この回路での役割    ; 起動時に内部VCCからBSTのコンデンサへ充電する低漏れダイオード。
      | ここでの動き        ; アノードをPV_DRV_VCC、カソードをPV_BSTへ接続する。BSTが上がった後は逆方向になり、浮いたBSTからVCCへ電荷が戻るのを抑える。
      | 部品を選ぶ理由      ; 200Vの小信号シリコンダイオード候補。逆漏れが小さいことを重視する。高温の漏れ電流もLTC7000Aの小さいチャージポンプ電流予算に影響する。
      | 定格と漏れの条件    ; 反復逆電圧200V、平均順電流200mA。逆漏れの最大例は125Vで25℃時1nA、150℃時3µA。異なる電圧や温度の保証と混同しない。
      | 保存モデル値        ; Vf=0.8 V、Ron=5 Ωの簡略2端子モデル。逆漏れ温度依存や全パルス特性の保証ではない。
      | 端子表現            ; 図はA/Kの2電気端子。SOT-23実パッケージの未使用端子・フットプリントはメーカー接続図に従う。
      | メーカー根拠        ; https://www.onsemi.com/pdf/datasheet/mmbd1501-d.pdf
      | 用語                ; BST：Bootstrap（高側駆動電源）。VCC：このIC内部の電源。A：Anode（アノード）、K：Cathode（カソード）。nA/µA：ナノアンペア/マイクロアンペア。
  PV_D_FLY : fl_lib/Electrical/Electrical Elements/Diode  Description=|  Vf=0.8 V  Ron=0.01 Ohm  Goff=1e-8 1/Ohm  i_specify=off  i_priority=None  i=0 A  i_nominal_specify=off  i_nominal_value=1  i_nominal_unit=A  v_specify=off  v_priority=None  v=0 V  v_nominal_specify=off  v_nominal_value=1  v_nominal_unit=V
      | この回路での名前    ; PV_D_FLY
      | 部品名              ; Vishay V20PW22-M3/I（候補）
      | この回路での役割    ; L2の電流が保護遮断直後も流れ続けるための迂回路を作り、正方向の過大電圧を抑えるダイオード。
      | ここでの動き        ; アノードA=PV_FILTERED、カソードK=PV_SENSED。通常時には逆方向で、遮断時などに必要な向きの電流帰路を作る。
      | 定格とその条件      ; 200V、20A級の単一ショットキーダイオード。20A定格はメーカーの放熱条件を伴う。今回の遮断パルス・反復・温度で安全と確認した意味ではない。
      | 実部品の端子        ; 実部品の1番と2番は両方ともアノード、放熱パッドKがカソード。図の標準DiodeはA/Kの2電気端子で、1番と2番の個別リードを描き分けていない。PCBでは両アノード端子とKパッドをメーカーのフットプリントどおり接続する。
      | 別部品にする理由    ; 各クランプのカソード電位が異なるため、通常の共通カソード2連ダイオード1個へそのまま置換できない。
      | 追加の設計意図      ; 
      | 保存モデル値        ; Vf=0.8 V、Ron=0.01 Ω。温度・逆漏れ・容量を含むメーカー完全モデルではない。
      | メーカー根拠        ; V20PW22: https://www.vishay.com/docs/87004/v20pw22.pdf 。TSの負電圧保護例: LTC7000A p.21 Fig.13 https://www.analog.com/media/en/technical-documentation/data-sheets/ltc7000a.pdf
      | 用語                ; A：Anode（アノード）。K：Cathode（カソード）。Vf：順電圧。Ron：導通中の抵抗近似。PCB：Printed Circuit Board（プリント基板）。ショットキーダイオード：金属と半導体の接合を使う整流素子。
  PV_D_GS : ee_lib/Semiconductors & Converters/Diode  Description=|  Vf=0.8 V  Ron=10 Ohm  Goff=4.7e-9 S  N_series=1  N_parallel=1  ZenerEnable=true  BV=15 V  Rz=15 Ohm  enable_fault_composite=simscape.enum.onoff.off  i_specify=off  i_priority=None  i=0 A  i_nominal_specify=off  i_nominal_value=1  i_nominal_unit=A  v_specify=off  v_priority=None  v=0 V  v_nominal_specify=off  v_nominal_value=1  v_nominal_unit=V  ModelType=ee.enum.diode.idealModelType.pwl  TableType=ee.enum.diode.tableType.IfMat  IfMat=[.07, .12, .19, 1.75, 4.24, 7.32, 11.2; .16, .3, .72, 2.14, 5.02, 8.35, 13.12] A  VfMat=[.9, 1.15, 1.25, 1.5, 1.75, 2.17, 2.6, 2.85; .58, .68, .75, 1.1, 1.38, 1.77, 2.27, 2.7] V  TjVec=[25, 125] degC  VfVec=[.5, .7, .9, 1.3, 1.7, 2.1, 2.5] V  IfVec=[.1, .2, .5, 1, 2, 4, 7, 10] A  IrMat=[1e-06, 2e-06, 5e-06, 1e-05, 2.5e-05, 5e-05, .0001; 2e-06, 5e-06, 1e-05, 4e-05, 8e-05, .0002, .0005] A  VrMat=[10, 100, 200, 250, 300, 325, 350; 10, 70, 160, 220, 270, 300, 320] V  VrVec=[10, 20, 40, 50, 70, 80, 100] V  IrVec=[1e-06, 2e-06, 5e-06, 1e-05, 2e-05, 5e-05, .0001] A  rec_loss_model=ee.enum.diode.reverseRecoveryModelTabulateUpTo3D.fixed  ErecVal=0 J  scaleWithIandV=true  ErecMat=zeros(2, 3) J  ErecMat3D=zeros(2, 3, 2) J  TjrecVec=[25, 125] degC  IfrecVec=[.1, 1, 10] A  IrecVal=10 A  VrecVal=10 V  VrecVec=[0, 100] V  tFilter=1 / 1000 / 100 s  thermal_network_parameterization=ee.enum.thermalNetworkTopology.junctionCase  Rth=[0, 10] K/W  Rth_Cauer=[1, 3, 10] K/W  Rth_Foster=[.08, .14, .22, .16] K/W  thermal_mass_parameterization=ee.enum.thermalNetwork.timeconstant  thermal_mass=[0, 1] J/K  thermal_mass_Cauer=[.1, .3, 1] J/K  thermal_mass_Foster=[.001, .005, .05, .5] J/K  thermal_time_constant=[0, 10] s  thermal_time_constant_Cauer=[1, 3, 10] s  thermal_time_constant_Foster=[7e-05, .0007, .01, .08] s  thermal_mass_initial_temperatures=[25, 25] degC  thermal_mass_initial_temperatures_Cauer=[25, 25, 25] degC  thermal_mass_initial_temperatures_Foster=[25, 25, 25, 25] degC  junction_thermal_mass=0.01 J/K  junction_temperature_specify=off  junction_temperature_priority=None  junction_temperature=25 degC  junction_temperature_nominal_specify=off  junction_temperature_nominal_value=1  junction_temperature_nominal_unit=degC  ThermalPort=false  ModelTypePhysical=ee.enum.diode.physicalModelType.exponential  prmExp=ee.enum.diode.expParam.useTwo  I12=[.0137, .545] A  V12=[.6, .7] V  IS=1e-12 A  ec=1  I1=0.0137 A  V1=0.6 V  RS=0 Ohm  C_param=ee.enum.diode.capParam.fixed  CJ=0 pF  CJ0=5 pF  Vvec=[.1, 10, 100] V  Cvec=[3.5, 1, .4] pF  VJ=1 V  Mgrad=0.5  FC=0.5  Q_param=ee.enum.diode.recoveryParam.off  iRM=-7.15 A  iF=4 A  didt=-750 A/us  trr_factor=3  trr=115 ns  Qrr=150 nA*s  Vr=-600 V  Ls=150 nH  Erec=0.03 J  TT=50 ns  tau=100 ns  T_param=ee.enum.diode.temperatureParam.off  Tmeas=25 degC  I1_T2=0.245 A  V1_T2=0.5 V  IS_T2=1.25e-7 A  Tmeas2=125 degC  EG_param=ee.enum.diode.egapParam.material_si  EG=1.11 eV  XTI_param=ee.enum.diode.xtiParam.pn  XTI=3  dBVdT=0 V/K  Tdevice=25 degC  i_capacitor_specify=off  i_capacitor_priority=None  i_capacitor=0 A  i_capacitor_nominal_specify=off  i_capacitor_nominal_value=1  i_capacitor_nominal_unit=A  Qj_specify=off  Qj_priority=None  Qj=0 C  Qj_nominal_specify=off  Qj_nominal_value=1  Qj_nominal_unit=uC
      | この回路での名前 ; PV_D_GS
      | 部品名 ; BZT52H-C15,115
      | 部品種別 ; 15 Vツェナーダイオード（共通ゲート保護）
      | ここでの役割 ; 出力短絡や過電流時に共通ソースが下がっても、ゲートとソース間の電圧が上がりすぎないよう電流を逃がす。2個のMOSFETの外部ゲートとソースが共通なので1個で保護する。
      | 端子と接続 ; 1 K（カソード）=PV_GATE、2 A（アノード）=PV_COMMON_SOURCE。
      | メーカー規定 ; 25 C、5 mAで13.8～15.6 V。微分抵抗は5 mAで最大15 Ohm、1 mAで最大110 Ohm。100 us単発のピーク逆電流は2 A。
      | モデル ; 標準Simscape DiodeのZenerモード。公称近似BV=15 V/Rz=15 Ohm。有限の傾きを持つ区分線形モデルであり、電流や温度によらず15 Vになる意味ではない。
      | 保守試験 ; BV=17.225 V/Rz=110 Ohmを別条件で確認する。これは高温と低電流域の仕様を組み合わせた工学的感度条件であり、メーカー保証の全域特性ではない。
      | 確認範囲 ; 追加しただけでは合格でない。内部VGS、ダイオード電流、損失、パルス幅を新しい試験で確認する。熱/SOA/実装寄生は別。
      | メーカー根拠 ; https://assets.nexperia.com/documents/data-sheet/BZT52H_SER.pdf
  PV_D_NEG : fl_lib/Electrical/Electrical Elements/Diode  Description=|  Vf=0.8 V  Ron=0.01 Ohm  Goff=1e-8 1/Ohm  i_specify=off  i_priority=None  i=0 A  i_nominal_specify=off  i_nominal_value=1  i_nominal_unit=A  v_specify=off  v_priority=None  v=0 V  v_nominal_specify=off  v_nominal_value=1  v_nominal_unit=V
      | この回路での名前    ; PV_D_NEG
      | 部品名              ; Vishay V20PW22-M3/I（候補）
      | この回路での役割    ; PV_FILTEREDがGNDより大きく負側へ振れるのを抑えるダイオード。
      | ここでの動き        ; アノードA=GND、カソードK=PV_FILTERED。通常時には逆方向で、遮断時などに必要な向きの電流帰路を作る。
      | 定格とその条件      ; 200V、20A級の単一ショットキーダイオード。20A定格はメーカーの放熱条件を伴う。今回の遮断パルス・反復・温度で安全と確認した意味ではない。
      | 実部品の端子        ; 実部品の1番と2番は両方ともアノード、放熱パッドKがカソード。図の標準DiodeはA/Kの2電気端子で、1番と2番の個別リードを描き分けていない。PCBでは両アノード端子とKパッドをメーカーのフットプリントどおり接続する。
      | 別部品にする理由    ; 各クランプのカソード電位が異なるため、通常の共通カソード2連ダイオード1個へそのまま置換できない。
      | 追加の設計意図      ; 
      | 保存モデル値        ; Vf=0.8 V、Ron=0.01 Ω。温度・逆漏れ・容量を含むメーカー完全モデルではない。
      | メーカー根拠        ; V20PW22: https://www.vishay.com/docs/87004/v20pw22.pdf 。TSの負電圧保護例: LTC7000A p.21 Fig.13 https://www.analog.com/media/en/technical-documentation/data-sheets/ltc7000a.pdf
      | 用語                ; A：Anode（アノード）。K：Cathode（カソード）。Vf：順電圧。Ron：導通中の抵抗近似。PCB：Printed Circuit Board（プリント基板）。ショットキーダイオード：金属と半導体の接合を使う整流素子。
  PV_D_TS : fl_lib/Electrical/Electrical Elements/Diode  Description=|  Vf=0.8 V  Ron=0.01 Ohm  Goff=1e-8 1/Ohm  i_specify=off  i_priority=None  i=0 A  i_nominal_specify=off  i_nominal_value=1  i_nominal_unit=A  v_specify=off  v_priority=None  v=0 V  v_nominal_specify=off  v_nominal_value=1  v_nominal_unit=V
      | この回路での名前    ; PV_D_TS
      | 部品名              ; Vishay V20PW22-M3/I（候補）
      | この回路での役割    ; 2個の保護MOSFETの共通ソースとLTC7000AのTS端子が負電圧へ振れすぎるのを抑えるダイオード。
      | ここでの動き        ; アノードA=GND、カソードK=PV_COMMON_SOURCE。通常時には逆方向で、遮断時などに必要な向きの電流帰路を作る。
      | 定格とその条件      ; 200V、20A級の単一ショットキーダイオード。20A定格はメーカーの放熱条件を伴う。今回の遮断パルス・反復・温度で安全と確認した意味ではない。
      | 実部品の端子        ; 実部品の1番と2番は両方ともアノード、放熱パッドKがカソード。図の標準DiodeはA/Kの2電気端子で、1番と2番の個別リードを描き分けていない。PCBでは両アノード端子とKパッドをメーカーのフットプリントどおり接続する。
      | 別部品にする理由    ; 各クランプのカソード電位が異なるため、通常の共通カソード2連ダイオード1個へそのまま置換できない。
      | 追加の設計意図      ; LTC7000AのTS負電圧対策の接続例を参考に、GNDからTSへ電流を供給する向きに置く。起動時に観測したTS負側変動への対策候補であり、この追加だけで全起動条件を保証しない。
      | 保存モデル値        ; Vf=0.8 V、Ron=0.01 Ω。温度・逆漏れ・容量を含むメーカー完全モデルではない。
      | メーカー根拠        ; V20PW22: https://www.vishay.com/docs/87004/v20pw22.pdf 。TSの負電圧保護例: LTC7000A p.21 Fig.13 https://www.analog.com/media/en/technical-documentation/data-sheets/ltc7000a.pdf
      | 用語                ; A：Anode（アノード）。K：Cathode（カソード）。Vf：順電圧。Ron：導通中の抵抗近似。PCB：Printed Circuit Board（プリント基板）。ショットキーダイオード：金属と半導体の接合を使う整流素子。
  PV_Q1 : ee_lib/Semiconductors & Converters/N-Channel MOSFET  Description=|  paramTerminal=ee.enum.mosfet.numberOfTerminals.three  parameterization=ee.enum.mosfet.parameterization.datasheet  Beta=5.0 A/V^2  Rds=0.0048 Ohm  Id=4 A  Vgs=10 V  Vth=4.1 V  Vth0=1.7 V  lam=0 1/V  gamma_vth=0.5 V^(1/2)  phib=0.5 V  Vth1=1.9071 V  Vbs1=-1 V  Vth2=2.066 V  Vbs2=-2 V  Tmeas=25 degC  Vgs_vec=[-1, -.5, 2, 3, 4, 5] V  Vds_vec=[0, 2, 4, 8, 12, 16, 20] V  Vbs_vec=[0, -4, -6, -12] V  T_vec=[25, 125] degC  Vth_vec=[.4, 1.2, 1.4, 1.45] V  Vth_mat=[.4, .35; 1.2, 1.15; 1.4, 1.35; 1.45, 1.4] V  Ids_mat=[0, 0, 0, 0, 0, 0, 0; 0, 0, 0, 0, 0, 0, 0; 0, .003, .0038, .0043, .0046, .0048, .0049; 0, .0055, .008, .009, .0095, .01, .0101; 0, .0115, .016, .018, .019, .0195, .02; 0, .0152, .0225, .0265, .028, .0295, .03] A  Ids_mat0=[0, 0, 0, 0, 0, 0, 0; 0, 0, 0, 0, 0, 0, 0; 0, .003, .0038, .0043, .0046, .0048, .0049; 0, .0055, .008, .009, .0095, .01, .0101; 0, .0115, .016, .018, .019, .0195, .02; 0, .0152, .0225, .0265, .028, .0295, .03] A  Ids_mat_3D=zeros(6, 7, 2) A  Ids_mat_3D0=zeros(6, 7, 2) A  IV_table_symmetry=ee.enum.mosfet.symmetricNIV.no  RS=0.0001 Ohm  RD=0.0001 Ohm  RB=0.001 Ohm  LeadRs=0 Ohm  LeadRd=0 Ohm  LeadRg=25 Ohm  LeadRb=0 Ohm  LS=0 nH  LD=0 nH  LG=0 nH  LB=0 nH  C_param=ee.enum.mosfet.capacitanceParam.fixedciss  C_GS=270 pF  C_GD=80 pF  C_GB=0 pF  C_DS=0 pF  C_iss=290e-12 F  C_rss=13e-12 F  C_oss=1400e-12 F  C_iss_vec=[720, 700, 590, 470, 390, 310] pF  C_rss_vec=[450, 400, 300, 190, 95, 55] pF  C_oss_vec=[900, 810, 690, 420, 270, 170] pF  C_GS_vec=[270, 300, 290, 280, 295, 255] pF  C_GD_vec=[450, 400, 300, 190, 95, 55] pF  C_GB_vec=[270, 300, 290, 280, 295, 255] pF  C_Vgs_vec=0 V  C_DS_vec=[450, 410, 390, 230, 175, 115] pF  C_Vds_vec=[.1, .3, 1, 3, 10, 30] V  V_GS_for_cap_data=0 V  charge_linearity_param=ee.enum.mosfet.cgdLinearity.constant  C_OX=200 pF  V_C_OX=-0.5 V  charge_linearity_param_vgb=ee.enum.mosfet.cgbLinearity.instantly  charge_linearity_param_with_vgb=ee.enum.mosfet.cgbLinearityWithSeparateCgb.instantly  Di_param=ee.enum.mosfet.diodeParam.exponential  IsDiode=1e-9 A  Vbi=0.6 V  n=1.5  Cj0Diode=0 pF  TT=0 s  Tmeas_dio=25 degC  TableTypeNoT=ee.enum.mosfet.tableType.IfMat  TableType=ee.enum.diode.tableType.IfMat  IfVec=[.07, .12, .19, 1.75, 4.24, 7.32, 11.2] A  IfMat=[.07, .12, .19, 1.75, 4.24, 7.32, 11.2; .16, .3, .72, 2.14, 4.02, 6.35, 9.12] A  VfVecV=[.9, 1.15, 1.25, 1.5, 1.75, 2.17, 2.6, 2.85] V  VfMatV=[.9, 1.15, 1.25, 1.5, 1.75, 2.17, 2.6, 2.85; .58, .68, .75, 1.1, 1.38, 1.77, 2.27, 2.7] V  TjVec=[25, 125] degC  VfVec=[.5, .7, .9, 1.3, 1.7, 2.1, 2.5] V  IfVecV=[.1, .2, .5, 1, 2, 4, 7, 10] A  diode_Goff=1e-12 1/Ohm  prmDatasheet=ee.enum.temperatureParameterization.none  prmEquCoeff=ee.enum.temperatureParameterization.none  dVth_dT=-6 mV/K  dVth0_dT=-6 mV/K  Rds_T2=0.037 Ohm  BEXDatasheet=-1.5  BEXEquCoeff=-1.5  etaisDatasheet=3  etaisEquCoeff=3  Tmeas2=125 degC  etaisTabulated=3  TdeviceDatasheet=25 degC  TdeviceEquCoeff=25 degC  TdeviceTabulated=25 degC  i_g_specify=off  i_g_priority=None  i_g=0 A  i_g_nominal_specify=off  i_g_nominal_value=1  i_g_nominal_unit=A  i_d_specify=off  i_d_priority=None  i_d=0 A  i_d_nominal_specify=off  i_d_nominal_value=1  i_d_nominal_unit=A  i_b_specify=off  i_b_priority=None  i_b=0 A  i_b_nominal_specify=off  i_b_nominal_value=1  i_b_nominal_unit=A  voltage_gs_specify=off  voltage_gs_priority=None  voltage_gs=0 V  voltage_gs_nominal_specify=off  voltage_gs_nominal_value=1  voltage_gs_nominal_unit=V  voltage_ds_specify=off  voltage_ds_priority=None  voltage_ds=0 V  voltage_ds_nominal_specify=off  voltage_ds_nominal_value=1  voltage_ds_nominal_unit=V  voltage_bs_specify=off  voltage_bs_priority=None  voltage_bs=0 V  voltage_bs_nominal_specify=off  voltage_bs_nominal_value=1  voltage_bs_nominal_unit=V  v_Cgs_specify=on  v_Cgs_priority=High  v_Cgs=0 V  v_Cgs_nominal_specify=off  v_Cgs_nominal_value=1  v_Cgs_nominal_unit=V  v_Cds_specify=off  v_Cds_priority=High  v_Cds=0 V  v_Cds_nominal_specify=off  v_Cds_nominal_value=1  v_Cds_nominal_unit=V  v_Cbs_specify=off  v_Cbs_priority=High  v_Cbs=0 V  v_Cbs_nominal_specify=off  v_Cbs_nominal_value=1  v_Cbs_nominal_unit=V  thermal_network_parameterization=ee.enum.thermalNetworkTopology.junctionCase  Rth=[0, 10] K/W  Rth_Cauer=[1, 3, 10] K/W  Rth_Foster=[.08, .14, .22, .16] K/W  thermal_mass_parameterization=ee.enum.thermalNetwork.timeconstant  thermal_mass=[0, 1] J/K  thermal_mass_Cauer=[.1, .3, 1] J/K  thermal_mass_Foster=[.001, .005, .05, .5] J/K  thermal_time_constant=[0, 10] s  thermal_time_constant_Cauer=[1, 3, 10] s  thermal_time_constant_Foster=[7e-05, .0007, .01, .08] s  thermal_mass_initial_temperatures=[25, 25] degC  thermal_mass_initial_temperatures_Cauer=[25, 25, 25] degC  Tvec_initial_Foster=[25, 25, 25, 25] degC  betaref=18 A/V^2  Vfbref=-1.1 V  gamma=3.5 V^(1/2)  phib2ref=1 V  thesatref=0.4 1/V  alpha=0  Vp=5e-2 V  thesrref=0 1/V  m=8  Tref=25 degC  Rsref=2e-3 Ohm  Rdref=0.17 Ohm  Rgref=8.4 Ohm  Rbref=2e-3 Ohm  Cox=1500 pF  Cgso=100 pF  Cgdo=14 pF  Isref=5.2e-13 A  Cj0=480 pF  Tprm=ee.enum.temperatureParameterization.none  etabet=1.3  Stvfb=5e-4 V/K  Stphib=-8.5e-4 V/K  etasat=1.04  etasr=0.65  etar=0.95  etais=3  Tsim=25 degC  Ig_specify=off  Ig_priority=None  Ig=0 A  Ig_nominal_specify=off  Ig_nominal_value=1  Ig_nominal_unit=nA  Ids_specify=off  Ids_priority=None  Ids=0 A  Ids_nominal_specify=off  Ids_nominal_value=1  Ids_nominal_unit=A  Ib_specify=off  Ib_priority=None  Ib=0 A  Ib_nominal_specify=off  Ib_nominal_value=1  Ib_nominal_unit=uA  V_gs_specify=off  V_gs_priority=None  V_gs=0 V  V_gs_nominal_specify=off  V_gs_nominal_value=1  V_gs_nominal_unit=V  V_ds_specify=off  V_ds_priority=None  V_ds=0 V  V_ds_nominal_specify=off  V_ds_nominal_value=1  V_ds_nominal_unit=V  V_bs_specify=off  V_bs_priority=None  V_bs=0 V  V_bs_nominal_specify=off  V_bs_nominal_value=1  V_bs_nominal_unit=V  QGoverCox_specify=off  QGoverCox_priority=None  QGoverCox=0 V  QGoverCox_nominal_specify=off  QGoverCox_nominal_value=1  QGoverCox_nominal_unit=V  QDoverCox_specify=off  QDoverCox_priority=None  QDoverCox=0 V  QDoverCox_nominal_specify=off  QDoverCox_nominal_value=1  QDoverCox_nominal_unit=V  QBoverCox_specify=off  QBoverCox_priority=None  QBoverCox=0 V  QBoverCox_nominal_specify=off  QBoverCox_nominal_value=1  QBoverCox_nominal_unit=V  T0=[25, 25] degC  T0_Cauer=[25, 25, 25] degC
      | この回路での名前    ; PV_Q1
      | 部品名              ; IPB048N15N5LFATMA1
      | この回路での役割    ; パネルと主電力段の間を開閉する保護用MOSFET。2個のソースを向かい合わせに接続し、OFF時に両方向の電流を遮断する構成。
      | ここでの動き        ; ドレインD=PV_FILTERED、ソースS=PV_COMMON_SOURCE、ゲートG=PV_GATE。LTC7000Aが共通ソースを基準にゲートを充放電する。主電力段のPWM用MOSFETとは別で、通電許可と保護停止に使う。
      | 表示と接続          ; Simscape標準MOSFETシンボル。G/D/Sの端子役割は保存モデルから引き継ぐ。図面を見やすく回転しても端子役割を入れ替えない。
      | 検証の範囲          ; この図面は実部品の端子と接続を示す。保存実行モジュール SHA256=f40bf5e1ef20bc97d0d4775a6ac457f3c30378c5fe9d07d29ab7bde4d975da32 の数値計算用ICコアを図面コピーから除去してある。実行用のICはメーカーのトランジスタモデルではなく、限定範囲の近似動作モデル。試験の合否と条件は C:\Users\hosik\OneDrive\ドキュメント\ChatGPT\oosem\evaluation\pv_protection_integration_20261023_r01\runtime\observations\standard_final_r04_aggregate\aggregate.json を参照する。
      | 実機への限界        ; メーカーの全トランジスタモデルではない。実部品のゲート電荷、寄生、温度、SOA、パルス耐量をこの図面だけで保証しない。
      | 用語                ; MOSFET：Metal-Oxide-Semiconductor Field-Effect Transistor（金属・酸化膜・半導体構造の電界効果トランジスタ）。G：Gate（ゲート）、D：Drain（ドレイン）、S：Source（ソース）。PWM：Pulse Width Modulation（パルス幅変調）。SOA：Safe Operating Area（安全動作領域）。
  PV_Q2 : ee_lib/Semiconductors & Converters/N-Channel MOSFET  Description=|  paramTerminal=ee.enum.mosfet.numberOfTerminals.three  parameterization=ee.enum.mosfet.parameterization.datasheet  Beta=5.0 A/V^2  Rds=0.0048 Ohm  Id=4 A  Vgs=10 V  Vth=4.1 V  Vth0=1.7 V  lam=0 1/V  gamma_vth=0.5 V^(1/2)  phib=0.5 V  Vth1=1.9071 V  Vbs1=-1 V  Vth2=2.066 V  Vbs2=-2 V  Tmeas=25 degC  Vgs_vec=[-1, -.5, 2, 3, 4, 5] V  Vds_vec=[0, 2, 4, 8, 12, 16, 20] V  Vbs_vec=[0, -4, -6, -12] V  T_vec=[25, 125] degC  Vth_vec=[.4, 1.2, 1.4, 1.45] V  Vth_mat=[.4, .35; 1.2, 1.15; 1.4, 1.35; 1.45, 1.4] V  Ids_mat=[0, 0, 0, 0, 0, 0, 0; 0, 0, 0, 0, 0, 0, 0; 0, .003, .0038, .0043, .0046, .0048, .0049; 0, .0055, .008, .009, .0095, .01, .0101; 0, .0115, .016, .018, .019, .0195, .02; 0, .0152, .0225, .0265, .028, .0295, .03] A  Ids_mat0=[0, 0, 0, 0, 0, 0, 0; 0, 0, 0, 0, 0, 0, 0; 0, .003, .0038, .0043, .0046, .0048, .0049; 0, .0055, .008, .009, .0095, .01, .0101; 0, .0115, .016, .018, .019, .0195, .02; 0, .0152, .0225, .0265, .028, .0295, .03] A  Ids_mat_3D=zeros(6, 7, 2) A  Ids_mat_3D0=zeros(6, 7, 2) A  IV_table_symmetry=ee.enum.mosfet.symmetricNIV.no  RS=0.0001 Ohm  RD=0.0001 Ohm  RB=0.001 Ohm  LeadRs=0 Ohm  LeadRd=0 Ohm  LeadRg=25 Ohm  LeadRb=0 Ohm  LS=0 nH  LD=0 nH  LG=0 nH  LB=0 nH  C_param=ee.enum.mosfet.capacitanceParam.fixedciss  C_GS=270 pF  C_GD=80 pF  C_GB=0 pF  C_DS=0 pF  C_iss=290e-12 F  C_rss=13e-12 F  C_oss=1400e-12 F  C_iss_vec=[720, 700, 590, 470, 390, 310] pF  C_rss_vec=[450, 400, 300, 190, 95, 55] pF  C_oss_vec=[900, 810, 690, 420, 270, 170] pF  C_GS_vec=[270, 300, 290, 280, 295, 255] pF  C_GD_vec=[450, 400, 300, 190, 95, 55] pF  C_GB_vec=[270, 300, 290, 280, 295, 255] pF  C_Vgs_vec=0 V  C_DS_vec=[450, 410, 390, 230, 175, 115] pF  C_Vds_vec=[.1, .3, 1, 3, 10, 30] V  V_GS_for_cap_data=0 V  charge_linearity_param=ee.enum.mosfet.cgdLinearity.constant  C_OX=200 pF  V_C_OX=-0.5 V  charge_linearity_param_vgb=ee.enum.mosfet.cgbLinearity.instantly  charge_linearity_param_with_vgb=ee.enum.mosfet.cgbLinearityWithSeparateCgb.instantly  Di_param=ee.enum.mosfet.diodeParam.exponential  IsDiode=1e-9 A  Vbi=0.6 V  n=1.5  Cj0Diode=0 pF  TT=0 s  Tmeas_dio=25 degC  TableTypeNoT=ee.enum.mosfet.tableType.IfMat  TableType=ee.enum.diode.tableType.IfMat  IfVec=[.07, .12, .19, 1.75, 4.24, 7.32, 11.2] A  IfMat=[.07, .12, .19, 1.75, 4.24, 7.32, 11.2; .16, .3, .72, 2.14, 4.02, 6.35, 9.12] A  VfVecV=[.9, 1.15, 1.25, 1.5, 1.75, 2.17, 2.6, 2.85] V  VfMatV=[.9, 1.15, 1.25, 1.5, 1.75, 2.17, 2.6, 2.85; .58, .68, .75, 1.1, 1.38, 1.77, 2.27, 2.7] V  TjVec=[25, 125] degC  VfVec=[.5, .7, .9, 1.3, 1.7, 2.1, 2.5] V  IfVecV=[.1, .2, .5, 1, 2, 4, 7, 10] A  diode_Goff=1e-12 1/Ohm  prmDatasheet=ee.enum.temperatureParameterization.none  prmEquCoeff=ee.enum.temperatureParameterization.none  dVth_dT=-6 mV/K  dVth0_dT=-6 mV/K  Rds_T2=0.037 Ohm  BEXDatasheet=-1.5  BEXEquCoeff=-1.5  etaisDatasheet=3  etaisEquCoeff=3  Tmeas2=125 degC  etaisTabulated=3  TdeviceDatasheet=25 degC  TdeviceEquCoeff=25 degC  TdeviceTabulated=25 degC  i_g_specify=off  i_g_priority=None  i_g=0 A  i_g_nominal_specify=off  i_g_nominal_value=1  i_g_nominal_unit=A  i_d_specify=off  i_d_priority=None  i_d=0 A  i_d_nominal_specify=off  i_d_nominal_value=1  i_d_nominal_unit=A  i_b_specify=off  i_b_priority=None  i_b=0 A  i_b_nominal_specify=off  i_b_nominal_value=1  i_b_nominal_unit=A  voltage_gs_specify=off  voltage_gs_priority=None  voltage_gs=0 V  voltage_gs_nominal_specify=off  voltage_gs_nominal_value=1  voltage_gs_nominal_unit=V  voltage_ds_specify=off  voltage_ds_priority=None  voltage_ds=0 V  voltage_ds_nominal_specify=off  voltage_ds_nominal_value=1  voltage_ds_nominal_unit=V  voltage_bs_specify=off  voltage_bs_priority=None  voltage_bs=0 V  voltage_bs_nominal_specify=off  voltage_bs_nominal_value=1  voltage_bs_nominal_unit=V  v_Cgs_specify=on  v_Cgs_priority=High  v_Cgs=0 V  v_Cgs_nominal_specify=off  v_Cgs_nominal_value=1  v_Cgs_nominal_unit=V  v_Cds_specify=off  v_Cds_priority=High  v_Cds=0 V  v_Cds_nominal_specify=off  v_Cds_nominal_value=1  v_Cds_nominal_unit=V  v_Cbs_specify=off  v_Cbs_priority=High  v_Cbs=0 V  v_Cbs_nominal_specify=off  v_Cbs_nominal_value=1  v_Cbs_nominal_unit=V  thermal_network_parameterization=ee.enum.thermalNetworkTopology.junctionCase  Rth=[0, 10] K/W  Rth_Cauer=[1, 3, 10] K/W  Rth_Foster=[.08, .14, .22, .16] K/W  thermal_mass_parameterization=ee.enum.thermalNetwork.timeconstant  thermal_mass=[0, 1] J/K  thermal_mass_Cauer=[.1, .3, 1] J/K  thermal_mass_Foster=[.001, .005, .05, .5] J/K  thermal_time_constant=[0, 10] s  thermal_time_constant_Cauer=[1, 3, 10] s  thermal_time_constant_Foster=[7e-05, .0007, .01, .08] s  thermal_mass_initial_temperatures=[25, 25] degC  thermal_mass_initial_temperatures_Cauer=[25, 25, 25] degC  Tvec_initial_Foster=[25, 25, 25, 25] degC  betaref=18 A/V^2  Vfbref=-1.1 V  gamma=3.5 V^(1/2)  phib2ref=1 V  thesatref=0.4 1/V  alpha=0  Vp=5e-2 V  thesrref=0 1/V  m=8  Tref=25 degC  Rsref=2e-3 Ohm  Rdref=0.17 Ohm  Rgref=8.4 Ohm  Rbref=2e-3 Ohm  Cox=1500 pF  Cgso=100 pF  Cgdo=14 pF  Isref=5.2e-13 A  Cj0=480 pF  Tprm=ee.enum.temperatureParameterization.none  etabet=1.3  Stvfb=5e-4 V/K  Stphib=-8.5e-4 V/K  etasat=1.04  etasr=0.65  etar=0.95  etais=3  Tsim=25 degC  Ig_specify=off  Ig_priority=None  Ig=0 A  Ig_nominal_specify=off  Ig_nominal_value=1  Ig_nominal_unit=nA  Ids_specify=off  Ids_priority=None  Ids=0 A  Ids_nominal_specify=off  Ids_nominal_value=1  Ids_nominal_unit=A  Ib_specify=off  Ib_priority=None  Ib=0 A  Ib_nominal_specify=off  Ib_nominal_value=1  Ib_nominal_unit=uA  V_gs_specify=off  V_gs_priority=None  V_gs=0 V  V_gs_nominal_specify=off  V_gs_nominal_value=1  V_gs_nominal_unit=V  V_ds_specify=off  V_ds_priority=None  V_ds=0 V  V_ds_nominal_specify=off  V_ds_nominal_value=1  V_ds_nominal_unit=V  V_bs_specify=off  V_bs_priority=None  V_bs=0 V  V_bs_nominal_specify=off  V_bs_nominal_value=1  V_bs_nominal_unit=V  QGoverCox_specify=off  QGoverCox_priority=None  QGoverCox=0 V  QGoverCox_nominal_specify=off  QGoverCox_nominal_value=1  QGoverCox_nominal_unit=V  QDoverCox_specify=off  QDoverCox_priority=None  QDoverCox=0 V  QDoverCox_nominal_specify=off  QDoverCox_nominal_value=1  QDoverCox_nominal_unit=V  QBoverCox_specify=off  QBoverCox_priority=None  QBoverCox=0 V  QBoverCox_nominal_specify=off  QBoverCox_nominal_value=1  QBoverCox_nominal_unit=V  T0=[25, 25] degC  T0_Cauer=[25, 25, 25] degC
      | この回路での名前    ; PV_Q2
      | 部品名              ; IPB048N15N5LFATMA1
      | この回路での役割    ; パネルと主電力段の間を開閉する保護用MOSFET。2個のソースを向かい合わせに接続し、OFF時に両方向の電流を遮断する構成。
      | ここでの動き        ; ドレインD=PV_OUT、ソースS=PV_COMMON_SOURCE、ゲートG=PV_GATE。LTC7000Aが共通ソースを基準にゲートを充放電する。主電力段のPWM用MOSFETとは別で、通電許可と保護停止に使う。
      | 表示と接続          ; Simscape標準MOSFETシンボル。G/D/Sの端子役割は保存モデルから引き継ぐ。図面を見やすく回転しても端子役割を入れ替えない。
      | 検証の範囲          ; この図面は実部品の端子と接続を示す。保存実行モジュール SHA256=f40bf5e1ef20bc97d0d4775a6ac457f3c30378c5fe9d07d29ab7bde4d975da32 の数値計算用ICコアを図面コピーから除去してある。実行用のICはメーカーのトランジスタモデルではなく、限定範囲の近似動作モデル。試験の合否と条件は C:\Users\hosik\OneDrive\ドキュメント\ChatGPT\oosem\evaluation\pv_protection_integration_20261023_r01\runtime\observations\standard_final_r04_aggregate\aggregate.json を参照する。
      | 実機への限界        ; メーカーの全トランジスタモデルではない。実部品のゲート電荷、寄生、温度、SOA、パルス耐量をこの図面だけで保証しない。
      | 用語                ; MOSFET：Metal-Oxide-Semiconductor Field-Effect Transistor（金属・酸化膜・半導体構造の電界効果トランジスタ）。G：Gate（ゲート）、D：Drain（ドレイン）、S：Source（ソース）。PWM：Pulse Width Modulation（パルス幅変調）。SOA：Safe Operating Area（安全動作領域）。
  PV_RAN : fl_lib/Electrical/Electrical Elements/Resistor  Description=|  R=100000 Ohm  i_specify=off  i_priority=None  i=0 A  i_nominal_specify=off  i_nominal_value=1  i_nominal_unit=A  v_specify=off  v_priority=None  v=0 V  v_nominal_specify=off  v_nominal_value=1  v_nominal_unit=V
      | この回路での名前    ; PV_RAN
      | 部品名              ; 未選定 / 100 kOhm
      | この回路での役割    ; 外部信号の開放時をLowにする仮値。
      | ここでの動き        ; ANALOG_OK と GND の間に配置。支援するIC近傍へ置く。
      | 公称値              ; 100 kOhm
      | 採用状態            ; 図面化のための候補定数。動作・SOA・熱・ノイズの成立から再調整する。
      | モデルの範囲        ; Simscape標準Resistor。型番の周波数依存・温度依存特性を同定したモデルではない。
      | 用語と選定の注意    ; 抵抗値・許容差・定格電圧・電力・温度範囲は部品選定時に照合する。
  PV_RFLT : fl_lib/Electrical/Electrical Elements/Resistor  Description=|  R=100 Ohm  i_specify=off  i_priority=None  i=0 A  i_nominal_specify=off  i_nominal_value=1  i_nominal_unit=A  v_specify=off  v_priority=None  v=0 V  v_nominal_specify=off  v_nominal_value=1  v_nominal_unit=V
      | この回路での名前    ; PV_RFLT
      | 部品名              ; 未選定 / 100 Ohm
      | この回路での役割    ; SNS-の短絡時電流を抑えるメーカー推奨の直列抵抗。
      | ここでの動き        ; PV_AFTER_SHUNT と PV_SNS_MINUS の間に配置。支援するIC近傍へ置く。
      | 公称値              ; 100 Ohm
      | 採用状態            ; 図面化のための候補定数。動作・SOA・熱・ノイズの成立から再調整する。
      | モデルの範囲        ; Simscape標準Resistor。型番の周波数依存・温度依存特性を同定したモデルではない。
      | 用語と選定の注意    ; 抵抗値・許容差・定格電圧・電力・温度範囲は部品選定時に照合する。
  PV_RFLT_PU : fl_lib/Electrical/Electrical Elements/Resistor  Description=|  R=22000 Ohm  i_specify=off  i_priority=None  i=0 A  i_nominal_specify=off  i_nominal_value=1  i_nominal_unit=A  v_specify=off  v_priority=None  v=0 V  v_nominal_specify=off  v_nominal_value=1  v_nominal_unit=V
      | この回路での名前    ; PV_RFLT_PU
      | 部品名              ; 未選定 / 22 kOhm
      | この回路での役割    ; FAULTオープンドレイン出力を3.3Vへプルアップする。
      | ここでの動き        ; P3V3 と OC_FAULT_N の間に配置。支援するIC近傍へ置く。
      | 公称値              ; 22 kOhm
      | 採用状態            ; 図面化のための候補定数。動作・SOA・熱・ノイズの成立から再調整する。
      | モデルの範囲        ; Simscape標準Resistor。型番の周波数依存・温度依存特性を同定したモデルではない。
      | 用語と選定の注意    ; 抵抗値・許容差・定格電圧・電力・温度範囲は部品選定時に照合する。
  PV_RG : fl_lib/Electrical/Electrical Elements/Resistor  Description=|  R=100000 Ohm  i_specify=off  i_priority=None  i=0 A  i_nominal_specify=off  i_nominal_value=1  i_nominal_unit=A  v_specify=off  v_priority=None  v=0 V  v_nominal_specify=off  v_nominal_value=1  v_nominal_unit=V
      | この回路での名前    ; PV_RG
      | 部品名              ; 型番未選定 / 保存定数を使用
      | この回路での役割    ; ON側のゲート充電を遅くする抵抗。追加のPV_C_SLEWと組み合わせ、突入電流を抑える。OFF側のTGDN経路を同じ抵抗で遅くする接続ではない。
      | 保存モデル値        ; R=100000
      | この図の範囲        ; この図面は実部品の端子と接続を示す。保存実行モジュール SHA256=f40bf5e1ef20bc97d0d4775a6ac457f3c30378c5fe9d07d29ab7bde4d975da32 の数値計算用ICコアを図面コピーから除去してある。実行用のICはメーカーのトランジスタモデルではなく、限定範囲の近似動作モデル。試験の合否と条件は C:\Users\hosik\OneDrive\ドキュメント\ChatGPT\oosem\evaluation\pv_protection_integration_20261023_r01\runtime\observations\standard_final_r04_aggregate\aggregate.json を参照する。
      | 注意                ; ゲート漏れ・チャージポンプの電流・起動時の電荷量・部品公差に依存する。値だけで突入や起動を保証しない。
  PV_RGS : fl_lib/Electrical/Electrical Elements/Resistor  Description=|  R=10000000 Ohm  i_specify=off  i_priority=None  i=0 A  i_nominal_specify=off  i_nominal_value=1  i_nominal_unit=A  v_specify=off  v_priority=None  v=0 V  v_nominal_specify=off  v_nominal_value=1  v_nominal_unit=V
      | この回路での名前    ; PV_RGS
      | 部品名              ; 未選定 / 10 MOhm
      | この回路での役割    ; ゲートとソース間の補助放電。12Vで1.2uA。チャージポンプの電流予算を圧迫しない高抵抗候補。
      | ここでの動き        ; PV_GATE と PV_COMMON_SOURCE の間に配置。支援するIC近傍へ置く。
      | 公称値              ; 10 MOhm
      | 採用状態            ; 図面化のための候補定数。動作・SOA・熱・ノイズの成立から再調整する。
      | モデルの範囲        ; Simscape標準Resistor。型番の周波数依存・温度依存特性を同定したモデルではない。
      | 用語と選定の注意    ; 抵抗値・許容差・定格電圧・電力・温度範囲は部品選定時に照合する。
  PV_RINP : fl_lib/Electrical/Electrical Elements/Resistor  Description=|  R=100000 Ohm  i_specify=off  i_priority=None  i=0 A  i_nominal_specify=off  i_nominal_value=1  i_nominal_unit=A  v_specify=off  v_priority=None  v=0 V  v_nominal_specify=off  v_nominal_value=1  v_nominal_unit=V
      | この回路での名前    ; PV_RINP
      | 部品名              ; 未選定 / 100 kOhm
      | この回路での役割    ; ドライバ入力が開放・ロジック電源停止したときLow側に置く。
      | ここでの動き        ; PV_ALLOW と GND の間に配置。支援するIC近傍へ置く。
      | 公称値              ; 100 kOhm
      | 採用状態            ; 図面化のための候補定数。動作・SOA・熱・ノイズの成立から再調整する。
      | モデルの範囲        ; Simscape標準Resistor。型番の周波数依存・温度依存特性を同定したモデルではない。
      | 用語と選定の注意    ; 抵抗値・許容差・定格電圧・電力・温度範囲は部品選定時に照合する。
  PV_ROV_H : fl_lib/Electrical/Electrical Elements/Resistor  Description=|  R=820000 Ohm  i_specify=off  i_priority=None  i=0 A  i_nominal_specify=off  i_nominal_value=1  i_nominal_unit=A  v_specify=off  v_priority=None  v=0 V  v_nominal_specify=off  v_nominal_value=1  v_nominal_unit=V
      | この回路での名前    ; PV_ROV_H
      | 部品名              ; 未選定 / 820 kOhm
      | この回路での役割    ; 入力過電圧しきい値の上側分圧抵抗。部品単体の定格電圧も確認する。
      | ここでの動き        ; PV_IN と PV_OV の間に配置。支援するIC近傍へ置く。
      | 公称値              ; 820 kOhm
      | 採用状態            ; 図面化のための候補定数。動作・SOA・熱・ノイズの成立から再調整する。
      | モデルの範囲        ; Simscape標準Resistor。型番の周波数依存・温度依存特性を同定したモデルではない。
      | 用語と選定の注意    ; 抵抗値・許容差・定格電圧・電力・温度範囲は部品選定時に照合する。
  PV_ROV_L : fl_lib/Electrical/Electrical Elements/Resistor  Description=|  R=10000 Ohm  i_specify=off  i_priority=None  i=0 A  i_nominal_specify=off  i_nominal_value=1  i_nominal_unit=A  v_specify=off  v_priority=None  v=0 V  v_nominal_specify=off  v_nominal_value=1  v_nominal_unit=V
      | この回路での名前    ; PV_ROV_L
      | 部品名              ; 未選定 / 10 kOhm
      | この回路での役割    ; OV停止公称100.43V、復帰92.13Vとなる仮値。
      | ここでの動き        ; PV_OV と GND の間に配置。支援するIC近傍へ置く。
      | 公称値              ; 10 kOhm
      | 採用状態            ; 図面化のための候補定数。動作・SOA・熱・ノイズの成立から再調整する。
      | モデルの範囲        ; Simscape標準Resistor。型番の周波数依存・温度依存特性を同定したモデルではない。
      | 用語と選定の注意    ; 抵抗値・許容差・定格電圧・電力・温度範囲は部品選定時に照合する。
  PV_RREARM : fl_lib/Electrical/Electrical Elements/Resistor  Description=|  R=100000 Ohm  i_specify=off  i_priority=None  i=0 A  i_nominal_specify=off  i_nominal_value=1  i_nominal_unit=A  v_specify=off  v_priority=None  v=0 V  v_nominal_specify=off  v_nominal_value=1  v_nominal_unit=V
      | この回路での名前    ; PV_RREARM
      | 部品名              ; 未選定 / 100 kOhm
      | この回路での役割    ; 外部信号の開放時をLowにする仮値。
      | ここでの動き        ; MCU_REARM と GND の間に配置。支援するIC近傍へ置く。
      | 公称値              ; 100 kOhm
      | 採用状態            ; 図面化のための候補定数。動作・SOA・熱・ノイズの成立から再調整する。
      | モデルの範囲        ; Simscape標準Resistor。型番の周波数依存・温度依存特性を同定したモデルではない。
      | 用語と選定の注意    ; 抵抗値・許容差・定格電圧・電力・温度範囲は部品選定時に照合する。
  PV_RREV_H : fl_lib/Electrical/Electrical Elements/Resistor  Description=|  R=10200 Ohm  i_specify=off  i_priority=None  i=0 A  i_nominal_specify=off  i_nominal_value=1  i_nominal_unit=A  v_specify=off  v_priority=None  v=0 V  v_nominal_specify=off  v_nominal_value=1  v_nominal_unit=V
      | この回路での名前    ; PV_RREV_H
      | 部品名              ; 未選定 / 10.2 kOhm 0.1%
      | この回路での役割    ; 逆流しきい値の上側分圧抵抗。
      | ここでの動き        ; VREF2V5 と V_REV の間に配置。支援するIC近傍へ置く。
      | 公称値              ; 10.2 kOhm 0.1%
      | 採用状態            ; 図面化のための候補定数。動作・SOA・熱・ノイズの成立から再調整する。
      | モデルの範囲        ; Simscape標準Resistor。型番の周波数依存・温度依存特性を同定したモデルではない。
      | 用語と選定の注意    ; 抵抗値・許容差・定格電圧・電力・温度範囲は部品選定時に照合する。
  PV_RREV_L : fl_lib/Electrical/Electrical Elements/Resistor  Description=|  R=9800 Ohm  i_specify=off  i_priority=None  i=0 A  i_nominal_specify=off  i_nominal_value=1  i_nominal_unit=A  v_specify=off  v_priority=None  v=0 V  v_nominal_specify=off  v_nominal_value=1  v_nominal_unit=V
      | この回路での名前    ; PV_RREV_L
      | 部品名              ; 未選定 / 9.8 kOhm 0.1%
      | この回路での役割    ; 分圧で公称1.225Vを作る。理想値では-0.5Aに対応する。
      | ここでの動き        ; V_REV と GND の間に配置。支援するIC近傍へ置く。
      | 公称値              ; 9.8 kOhm 0.1%
      | 採用状態            ; 図面化のための候補定数。動作・SOA・熱・ノイズの成立から再調整する。
      | モデルの範囲        ; Simscape標準Resistor。型番の周波数依存・温度依存特性を同定したモデルではない。
      | 用語と選定の注意    ; 抵抗値・許容差・定格電圧・電力・温度範囲は部品選定時に照合する。
  PV_RRUN : fl_lib/Electrical/Electrical Elements/Resistor  Description=|  R=100000 Ohm  i_specify=off  i_priority=None  i=0 A  i_nominal_specify=off  i_nominal_value=1  i_nominal_unit=A  v_specify=off  v_priority=None  v=0 V  v_nominal_specify=off  v_nominal_value=1  v_nominal_unit=V
      | この回路での名前    ; PV_RRUN
      | 部品名              ; 未選定 / 100 kOhm
      | この回路での役割    ; 外部信号の開放時をLowにする仮値。
      | ここでの動き        ; MCU_RUN と GND の間に配置。支援するIC近傍へ置く。
      | 公称値              ; 100 kOhm
      | 採用状態            ; 図面化のための候補定数。動作・SOA・熱・ノイズの成立から再調整する。
      | モデルの範囲        ; Simscape標準Resistor。型番の周波数依存・温度依存特性を同定したモデルではない。
      | 用語と選定の注意    ; 抵抗値・許容差・定格電圧・電力・温度範囲は部品選定時に照合する。
  PV_RTIME : fl_lib/Electrical/Electrical Elements/Resistor  Description=|  R=100000 Ohm  i_specify=off  i_priority=None  i=0 A  i_nominal_specify=off  i_nominal_value=1  i_nominal_unit=A  v_specify=off  v_priority=None  v=0 V  v_nominal_specify=off  v_nominal_value=1  v_nominal_unit=V
      | この回路での名前    ; PV_RTIME
      | 部品名              ; 未選定 / 100 kOhm
      | この回路での役割    ; TIMERの自動再試行を抑え、過電流後の停止を保持するメーカー回路例。
      | ここでの動き        ; PV_TIMER と GND の間に配置。支援するIC近傍へ置く。
      | 公称値              ; 100 kOhm
      | 採用状態            ; 図面化のための候補定数。動作・SOA・熱・ノイズの成立から再調整する。
      | モデルの範囲        ; Simscape標準Resistor。型番の周波数依存・温度依存特性を同定したモデルではない。
      | 用語と選定の注意    ; 抵抗値・許容差・定格電圧・電力・温度範囲は部品選定時に照合する。
  PV_RUV_H : fl_lib/Electrical/Electrical Elements/Resistor  Description=|  R=330000 Ohm  i_specify=off  i_priority=None  i=0 A  i_nominal_specify=off  i_nominal_value=1  i_nominal_unit=A  v_specify=off  v_priority=None  v=0 V  v_nominal_specify=off  v_nominal_value=1  v_nominal_unit=V
      | この回路での名前    ; PV_RUV_H
      | 部品名              ; 未選定 / 330 kOhm
      | この回路での役割    ; 入力低電圧しきい値の上側分圧抵抗。部品単体の定格電圧も確認する。
      | ここでの動き        ; PV_IN と PV_RUN_UV の間に配置。支援するIC近傍へ置く。
      | 公称値              ; 330 kOhm
      | 採用状態            ; 図面化のための候補定数。動作・SOA・熱・ノイズの成立から再調整する。
      | モデルの範囲        ; Simscape標準Resistor。型番の周波数依存・温度依存特性を同定したモデルではない。
      | 用語と選定の注意    ; 抵抗値・許容差・定格電圧・電力・温度範囲は部品選定時に照合する。
  PV_RUV_L : fl_lib/Electrical/Electrical Elements/Resistor  Description=|  R=10200 Ohm  i_specify=off  i_priority=None  i=0 A  i_nominal_specify=off  i_nominal_value=1  i_nominal_unit=A  v_specify=off  v_priority=None  v=0 V  v_nominal_specify=off  v_nominal_value=1  v_nominal_unit=V
      | この回路での名前    ; PV_RUV_L
      | 部品名              ; 未選定 / 10.2 kOhm
      | この回路での役割    ; UV開始公称約40.36V、停止約37.02Vとなる仮値。
      | ここでの動き        ; PV_RUN_UV と GND の間に配置。支援するIC近傍へ置く。
      | 公称値              ; 10.2 kOhm
      | 採用状態            ; 図面化のための候補定数。動作・SOA・熱・ノイズの成立から再調整する。
      | モデルの範囲        ; Simscape標準Resistor。型番の周波数依存・温度依存特性を同定したモデルではない。
      | 用語と選定の注意    ; 抵抗値・許容差・定格電圧・電力・温度範囲は部品選定時に照合する。
  PV_RVCCUV : fl_lib/Electrical/Electrical Elements/Resistor  Description=|  R=113000 Ohm  i_specify=off  i_priority=None  i=0 A  i_nominal_specify=off  i_nominal_value=1  i_nominal_unit=A  v_specify=off  v_priority=None  v=0 V  v_nominal_specify=off  v_nominal_value=1  v_nominal_unit=V
      | この回路での名前    ; PV_RVCCUV
      | 部品名              ; 未選定 / 113 kOhm
      | この回路での役割    ; ゲート駆動電源のUVLOを公称約7.91Vへ設定する仮値。
      | ここでの動き        ; PV_VCCUV と GND の間に配置。支援するIC近傍へ置く。
      | 公称値              ; 113 kOhm
      | 採用状態            ; 図面化のための候補定数。動作・SOA・熱・ノイズの成立から再調整する。
      | モデルの範囲        ; Simscape標準Resistor。型番の周波数依存・温度依存特性を同定したモデルではない。
      | 用語と選定の注意    ; 抵抗値・許容差・定格電圧・電力・温度範囲は部品選定時に照合する。
  PV_R_SLEW : fl_lib/Electrical/Electrical Elements/Resistor  Description=|  R=10 Ohm  i_specify=off  i_priority=None  i=0 A  i_nominal_specify=off  i_nominal_value=1  i_nominal_unit=A  v_specify=off  v_priority=None  v=0 V  v_nominal_specify=off  v_nominal_value=1  v_nominal_unit=V
      | この回路での名前    ; PV_R_SLEW
      | 部品名              ; 型番未選定 / 10 Ω
      | この回路での役割    ; ゲートの傾きを設定する追加コンデンサへ急な電流が集中しにくくする直列抵抗。
      | ここでの動き        ; 10Ω。PV_C_SLEWの直近へ置く。PV_RGの100kΩとは別の役割。
      | 端子と接続          ; PV_GATE と PV_SLEW の間
      | 保存モデル値        ; R=10
      | 選定の範囲          ; 保存モデルの定数を表す。実部品の型番・公差・電力・温度・周波数依存の最終選定は別。ここではモデルの値や接続を変更していない。
      | メーカー根拠        ; LTC7000A Fig.12: https://www.analog.com/media/en/technical-documentation/data-sheets/ltc7000a.pdf 。TPS3704: https://www.ti.com/lit/ds/symlink/tps3704.pdf
      | 用語                ; MLCC：Multilayer Ceramic Capacitor（積層セラミックコンデンサ）。DC：Direct Current（直流）。バイパス容量はICの切替時に生じる高周波電流の局所帰路を作る。狙う周波数は容量だけでなく実効容量・ESR（等価直列抵抗）・ESL（等価直列インダクタンス）と配置で決まる。
  PV_R_SUP25 : fl_lib/Electrical/Electrical Elements/Resistor  Description=|  R=21300 Ohm  i_specify=off  i_priority=None  i=0 A  i_nominal_specify=off  i_nominal_value=1  i_nominal_unit=A  v_specify=off  v_priority=None  v=0 V  v_nominal_specify=off  v_nominal_value=1  v_nominal_unit=V
      | この回路での名前    ; PV_R_SUP25
      | 部品名              ; 型番未選定 / 21.3 kΩ
      | この回路での役割    ; 2.5V基準監視の上側分圧抵抗。
      | ここでの動き        ; PV_U6のSENSE2近傍へ置き、PV_R_SUP26と組にする。
      | 端子と接続          ; VREF2V5 と PV_SUP_2V5 の間
      | 保存モデル値        ; R=21300
      | 選定の範囲          ; 保存モデルの定数を表す。実部品の型番・公差・電力・温度・周波数依存の最終選定は別。ここではモデルの値や接続を変更していない。
      | メーカー根拠        ; LTC7000A Fig.12: https://www.analog.com/media/en/technical-documentation/data-sheets/ltc7000a.pdf 。TPS3704: https://www.ti.com/lit/ds/symlink/tps3704.pdf
      | 用語                ; MLCC：Multilayer Ceramic Capacitor（積層セラミックコンデンサ）。DC：Direct Current（直流）。バイパス容量はICの切替時に生じる高周波電流の局所帰路を作る。狙う周波数は容量だけでなく実効容量・ESR（等価直列抵抗）・ESL（等価直列インダクタンス）と配置で決まる。
  PV_R_SUP26 : fl_lib/Electrical/Electrical Elements/Resistor  Description=|  R=10000 Ohm  i_specify=off  i_priority=None  i=0 A  i_nominal_specify=off  i_nominal_value=1  i_nominal_unit=A  v_specify=off  v_priority=None  v=0 V  v_nominal_specify=off  v_nominal_value=1  v_nominal_unit=V
      | この回路での名前    ; PV_R_SUP26
      | 部品名              ; 型番未選定 / 10 kΩ
      | この回路での役割    ; 2.5V基準監視の下側分圧抵抗。
      | ここでの動き        ; PV_U6のSENSE2近傍へ置き、PV_R_SUP25と組にする。
      | 端子と接続          ; PV_SUP_2V5 と GND の間
      | 保存モデル値        ; R=10000
      | 選定の範囲          ; 保存モデルの定数を表す。実部品の型番・公差・電力・温度・周波数依存の最終選定は別。ここではモデルの値や接続を変更していない。
      | メーカー根拠        ; LTC7000A Fig.12: https://www.analog.com/media/en/technical-documentation/data-sheets/ltc7000a.pdf 。TPS3704: https://www.ti.com/lit/ds/symlink/tps3704.pdf
      | 用語                ; MLCC：Multilayer Ceramic Capacitor（積層セラミックコンデンサ）。DC：Direct Current（直流）。バイパス容量はICの切替時に生じる高周波電流の局所帰路を作る。狙う周波数は容量だけでなく実効容量・ESR（等価直列抵抗）・ESL（等価直列インダクタンス）と配置で決まる。
  PV_R_SUP31 : fl_lib/Electrical/Electrical Elements/Resistor  Description=|  R=31200 Ohm  i_specify=off  i_priority=None  i=0 A  i_nominal_specify=off  i_nominal_value=1  i_nominal_unit=A  v_specify=off  v_priority=None  v=0 V  v_nominal_specify=off  v_nominal_value=1  v_nominal_unit=V
      | この回路での名前    ; PV_R_SUP31
      | 部品名              ; 型番未選定 / 31.2 kΩ
      | この回路での役割    ; 3.3V監視の上側分圧抵抗。
      | ここでの動き        ; PV_U6のSENSE1近傍へ置き、PV_R_SUP32と組にする。
      | 端子と接続          ; P3V3 と PV_SUP_3V3 の間
      | 保存モデル値        ; R=31200
      | 選定の範囲          ; 保存モデルの定数を表す。実部品の型番・公差・電力・温度・周波数依存の最終選定は別。ここではモデルの値や接続を変更していない。
      | メーカー根拠        ; LTC7000A Fig.12: https://www.analog.com/media/en/technical-documentation/data-sheets/ltc7000a.pdf 。TPS3704: https://www.ti.com/lit/ds/symlink/tps3704.pdf
      | 用語                ; MLCC：Multilayer Ceramic Capacitor（積層セラミックコンデンサ）。DC：Direct Current（直流）。バイパス容量はICの切替時に生じる高周波電流の局所帰路を作る。狙う周波数は容量だけでなく実効容量・ESR（等価直列抵抗）・ESL（等価直列インダクタンス）と配置で決まる。
  PV_R_SUP32 : fl_lib/Electrical/Electrical Elements/Resistor  Description=|  R=10000 Ohm  i_specify=off  i_priority=None  i=0 A  i_nominal_specify=off  i_nominal_value=1  i_nominal_unit=A  v_specify=off  v_priority=None  v=0 V  v_nominal_specify=off  v_nominal_value=1  v_nominal_unit=V
      | この回路での名前    ; PV_R_SUP32
      | 部品名              ; 型番未選定 / 10 kΩ
      | この回路での役割    ; 3.3V監視の下側分圧抵抗。
      | ここでの動き        ; PV_U6のSENSE1近傍へ置き、PV_R_SUP31と組にする。
      | 端子と接続          ; PV_SUP_3V3 と GND の間
      | 保存モデル値        ; R=10000
      | 選定の範囲          ; 保存モデルの定数を表す。実部品の型番・公差・電力・温度・周波数依存の最終選定は別。ここではモデルの値や接続を変更していない。
      | メーカー根拠        ; LTC7000A Fig.12: https://www.analog.com/media/en/technical-documentation/data-sheets/ltc7000a.pdf 。TPS3704: https://www.ti.com/lit/ds/symlink/tps3704.pdf
      | 用語                ; MLCC：Multilayer Ceramic Capacitor（積層セラミックコンデンサ）。DC：Direct Current（直流）。バイパス容量はICの切替時に生じる高周波電流の局所帰路を作る。狙う周波数は容量だけでなく実効容量・ESR（等価直列抵抗）・ESL（等価直列インダクタンス）と配置で決まる。
  PV_R_SUP_PU : fl_lib/Electrical/Electrical Elements/Resistor  Description=|  R=10000 Ohm  i_specify=off  i_priority=None  i=0 A  i_nominal_specify=off  i_nominal_value=1  i_nominal_unit=A  v_specify=off  v_priority=None  v=0 V  v_nominal_specify=off  v_nominal_value=1  v_nominal_unit=V
      | この回路での名前    ; PV_R_SUP_PU
      | 部品名              ; 型番未選定 / 10 kΩ
      | この回路での役割    ; 2本のRESETが解放されたときANALOG_OKをHighへ上げるプルアップ抵抗。
      | ここでの動き        ; PV_U6のRESET接続点の近傍へ置く。どちらかの出力がLowへ引けばANALOG_OKもLowになる。
      | 端子と接続          ; P3V3 と ANALOG_OK の間
      | 保存モデル値        ; R=10000
      | 選定の範囲          ; 保存モデルの定数を表す。実部品の型番・公差・電力・温度・周波数依存の最終選定は別。ここではモデルの値や接続を変更していない。
      | メーカー根拠        ; LTC7000A Fig.12: https://www.analog.com/media/en/technical-documentation/data-sheets/ltc7000a.pdf 。TPS3704: https://www.ti.com/lit/ds/symlink/tps3704.pdf
      | 用語                ; MLCC：Multilayer Ceramic Capacitor（積層セラミックコンデンサ）。DC：Direct Current（直流）。バイパス容量はICの切替時に生じる高周波電流の局所帰路を作る。狙う周波数は容量だけでなく実効容量・ESR（等価直列抵抗）・ESL（等価直列インダクタンス）と配置で決まる。
  PV_U1 : Subsystem  Description=|
      | この回路での名前    ; PV_U1
      | 部品名              ; LTC7000ARMSE#PBF
      | この回路での役割    ; パネル側の遮断用MOSFET 2個を動かす保護付きゲートドライバ。
      | ここでの動き        ; PV_ALLOWがHighで、入力電圧・駆動電源・ブートストラップ電源が成立し、保護が作動していない場合に2個のMOSFETをONへ向ける。LowではTGDNを通してゲートを共通ソースへ放電する。順方向過電流と入力UV/OVはこのICが担当し、逆流判定そのものはPV_U3が担当する。内部VCCを作り、BSTからゲートへ電荷を供給する。
      | 読み取りの注意      ; RUN端子のPV_RUN_UVは抵抗分圧による低電圧判定で、MCU_RUN信号とは別。R27=1mΩ、ISET=GNDの公称過電流検出は約20Aであり、15Aで必ず停止する設定ではない。UV/OVも公称約40V/100Vで、公差・遅延を含む実際の停止範囲は試験条件を参照する。BSTの対GND電圧とBST−TSの両方を確認する。IMONは意図的に未使用。
      | 端子と接続          ; 1 RUN → PV_RUN_UV、2 VIN → PV_IN、3 VCC → PV_DRV_VCC、4 VCCUV → PV_VCCUV、5 FAULT_N → OC_FAULT_N、6 TIMER → PV_TIMER、7 INP → PV_ALLOW、8 OVLO → PV_OV、16 SNS+ → PV_IN、15 SNS- → PV_SNS_MINUS、14 BST → PV_BST、13 TS → PV_COMMON_SOURCE、12 TGUP → PV_GATE_UP、11 TGDN → PV_GATE、10 IMON → NC（IMON未使用）、9 ISET → GND、17 GND → GND
      | パッケージと視点    ; MSE16 + exposed pad17。メーカー上面図の物理番号順。LTC7000Aの17番露出パッドは実物では裏面、図面では左下へ引き出す。
      | この図の範囲        ; この図面は実部品の端子と接続を示す。保存実行モジュール SHA256=f40bf5e1ef20bc97d0d4775a6ac457f3c30378c5fe9d07d29ab7bde4d975da32 の数値計算用ICコアを図面コピーから除去してある。実行用のICはメーカーのトランジスタモデルではなく、限定範囲の近似動作モデル。試験の合否と条件は C:\Users\hosik\OneDrive\ドキュメント\ChatGPT\oosem\evaluation\pv_protection_integration_20261023_r01\runtime\observations\standard_final_r04_aggregate\aggregate.json を参照する。
      | ソフトウェア確認    ; 試験で与えた指令・境界条件と、RP2040上で動くMicroPythonプログラムの実行確認は別。今回の記述は実ファームウェアの動作試験を実施したという意味ではない。
      | メーカー根拠        ; https://www.analog.com/media/en/technical-documentation/data-sheets/ltc7000a.pdf
      | 回路は変更していません。現在の **PV_U1＝LTC7000A（LTC7000ARMSE#PBF）**について、今の接続に沿って説明します。
      | このICは、パネル側の保護MOSFETを開閉し、電圧や電流の条件が悪ければ停止させる部品です。充電用の大電流は外付けMOSFETを通り、ICはそのゲートを操作します。内部に電源回路とチャージポンプがあり、MOSFETをONのまま維持できます。メーカー製品説明
      | 以下の数値は、仕様書の代表値と現在の抵抗・コンデンサから求めた目安です。実機での保証値ではありません。
      | まず、電圧の基準が２つあります。
      | 制御信号や電源入力は共通GND基準です。一方、ゲート駆動は TSにつながるMOSFETのソースを基準にします。この違いが特に重要です。
      | 1番 RUN：パネル電圧が十分になったら動作を許可する
      | 現回路では、パネル電圧を 330 kΩと10.2 kΩで小さくした電圧が入ります。
      | RUNが上昇して約1.21 Vを超えると動作許可、低下して約1.1 Vを下回ると停止です。現在の抵抗値では、パネル側に換算して約40.4 Vで許可、約37 Vまで下がると停止になります。
      | 起動と停止の電圧を離すことで、境界付近でON/OFFを繰り返しにくくしています。これを「ヒステリシス」と呼びます。
      | なお、RUNが約0.7 Vを超えると内部電源が動き始めますが、この段階ではまだゲートのONは許可されません。
      | 2番 VIN：このIC自身が動くための電力を受け取る
      | 現回路では、パネル側の PV_INにつながっています。
      | このICの低電圧電源は、ここから内部で作ります。 現在の構成では、別の12 V電源を外から引き込む必要はありません。端子付近の100 nFコンデンサは電源の急な変動を抑えるためのものです。
      | 14 Aなどの充電電流を、この端子に流し込むわけではありません。
      | 3番 VCC：内部で作った約10 Vが現れる端子
      | VINから内部の電圧調整回路で作られた、IC内部とゲート駆動回路のための電源です。現回路では1 µFのコンデンサがGNDとの間にあります。
      | VINが十分高いとき、おおむね10 Vになります。このVCCは、後述するBST側への初期充電にも使っています。
      | 今の接続では「外から12 Vを入れている端子」ではなく、内部で作った電源を外付けコンデンサで安定させている端子です。
      | 4番 VCCUV：内部電源が弱すぎる状態で、MOSFETをONさせないための設定
      | UVは低電圧を意味します。
      | 現回路では 113 kΩを介してGNDへ接続しています。この抵抗値によって、VCCが上昇したときの動作許可条件を約7.91 Vに設定しています。
      | つまり、パネル電圧の条件をRUNが満たしていても、ゲート駆動用の電源がまだ十分でなければONを待ちます。この端子が7.91 Vを作るのではなく、「VCCを何V以上で使い始めるか」を設定しています。
      | 以上の電源・低電圧判定の仕様は、仕様書p.9、18～19にあります。
      | 5番 FAULT：過電流などによる停止を外部へ知らせる
      | 図では FAULT_N → OC_FAULT_Nとなっています。末尾のNは、Low側で通知が有効になる意味です。
      | 現回路では22 kΩで3.3 Vへ引き上げています。ICが異常を通知すると、この線をLowへ引き下げます。
      | 過電流の場合は、後述するTIMERの電圧が約1.3 Vになると通知し、約1.4 Vでゲートを停止させます。つまり、少し先に通知が出ます。
      | Highだから保護回路のすべてが正常、あるいはMOSFETがONだと確認できる端子ではありません。
      | 6番 TIMER：過電流がどのくらい続いたら停止するかを決める
      | 現回路では 1 nFと100 kΩを並列にしてGNDへ接続しています。
      | 過電流を検出すると、ICがコンデンサを充電します。その電圧が停止しきい値に届くと、MOSFETをOFFにします。
      | 今の値では、継続する過電流に対して停止指令まで十数µs、計算上は約17 µs程度が目安です。そこからゲートが放電され、主電流が減るまでの時間は別にあります。
      | 並列の100 kΩには、過電流停止後の自動再試行を禁止する役割があります。再開にはINPをいったんLowにし、再度Highにする操作が必要です。
      | 7番 INP：外部から「保護MOSFETをONにしてよい」と指示する
      | 現回路では PV_ALLOWにつながっています。逆流判定などをまとめた外部の許可回路から指示を受けます。
      | 0 V：OFF指示
      | 3.3 V：ON要求
      | ON要求があっても、RUN、VCC、OVLO、過電流停止などの条件を満たさなければONにはなりません。
      | 100 kΩのプルダウン抵抗によって、外部回路が信号を出せない間はLow側に寄せています。ここで扱うのはパネル保護スイッチの開閉指令です。
      | 8番 OVLO：パネル電圧が高すぎると停止する
      | OVLOは「過電圧による動作禁止」です。
      | 現回路では、パネル電圧を 820 kΩと10 kΩで分圧して入れています。現在の値では、パネル電圧が約100.4 Vまで上がると停止し、約91～92 Vまで下がると過電圧による禁止が解除される計算です。
      | これは、電圧を100 Vに調整する機能ではありません。保護MOSFETをOFFにする機能です。また、過電圧が解除されても、ほかの条件が成立しなければONには戻りません。
      | 9番 ISET：過電流の判定基準を設定する
      | 現回路では GNDへ接続しています。この接続では、SNS端子間の電圧差が代表値で約20 mVになると過電流と判定します。
      | 電流検出抵抗R27は1 mΩなので、基本の計算は、
      | \[ 20\ \mathrm{mV} \div 1\ \mathrm{m\Omega}=20\ \mathrm{A} \]
      | です。現在のSNS−側の100 ΩとIC入力電流の影響まで入れると、代表値で約19.6 Aになります。
      | ただし、ICの判定電圧自体にばらつきがあるため、19.6 Aぴったりで遮断する設定ではありません。 また、この機能は電流を20 Aに調整して流し続ける制御ではなく、過電流を検出して停止させる保護です。
      | 10番 IMON：検出した電流を電圧として外へ出す
      | IMONは電流監視用の出力です。SNS端子間の電圧差を、おおむね20倍した電圧を出します。
      | R27が1 mΩなら、誤差を省いた例では10 Aで約0.2 Vです。
      | 現回路では未接続です。電流測定には別の測定回路を使っています。この出力だけで、停止中も含む双方向の電流測定ができるとは扱っていません。
      | 保護条件と電流監視の詳細は、仕様書p.5、9～10、15～18にあります。
      | 11番 TGDN：ゲートから電荷を抜いて、MOSFETをOFFにする
      | 現回路では、保護MOSFET PV_Q1とPV_Q2の共通ゲートに直接つながっています。
      | OFFにするとき、ゲートをTSと同じ電位へ引き下げます。 ゲートとソースの電圧差がほぼ0 Vになることで、MOSFETがOFFになります。
      | 例えばソースが80 Vなら、ゲートも約80 Vに下げます。共通GNDの0 Vまで引き下げる動作ではありません。
      | 12番 TGUP：ゲートへ電荷を入れて、MOSFETをONにする
      | 現回路では 100 kΩのPV_RGを通して、同じ共通ゲートへつながっています。
      | この抵抗と周辺のコンデンサによって、ONへ移る速度を抑えています。一方、OFF側のTGDNはこの100 kΩを通らず、直接ゲートを放電できます。
      | TGUPとTGDNは、２個のMOSFETを別々に操作する２チャンネルではありません。同じゲートを「充電する経路」と「放電する経路」です。
      | 13番 TS：ゲート駆動の基準となる、MOSFETのソース電位を受け取る
      | 現回路では、保護MOSFET２個の共通ソースである PV_COMMON_SOURCEにつながっています。
      | ICはこの電位を基準にして、ゲートを上げ下げします。
      | 
      | TSの電圧が80 Vの場合
      | ゲート電圧の例
      | ゲート－ソース間
      | ON
      | 約92 V
      | 約12 V
      | OFF
      | 約80 V
      | 約0 V
      | 
      | これは動作の説明用の例です。TSは共通GNDでも、主電力段のSWでもありません。
      | 14番 BST：TSより高いゲート駆動電圧を蓄える
      | 現回路では、BSTとTSの間に10 µFがあります。このコンデンサが、ゲートをONにするための電力を蓄えます。
      | 着目する電圧は BST－TSで、通常は約12 Vが目安です。BSTがGNDに対して常に12 Vという意味ではありません。
      | VCCからのダイオードは初期充電を助けます。その後も内部チャージポンプが電圧を維持するため、保護MOSFETをONのまま保持できます。
      | 15番 SNS−：電流検出抵抗の下流側の電圧を読む
      | 現回路では、R27の下流側から100 ΩのPV_RFLTを通して接続しています。
      | 次のSNS+と組み合わせ、R27でどれだけ電圧が下がったかを調べます。名前の「−」は、比較する２点のうち下流側という意味です。GND端子ではありません。
      | 16番 SNS+：電流検出抵抗の上流側の電圧を読む
      | 現回路では、R27よりパネル側のPV_INにつながっています。
      | 例えばR27の上流が80.000 V、下流が79.986 Vなら、抵抗両端の差は14 mVです。R27が1 mΩなので、ここから14 Aと判断できます。
      | このICは、その差がISETで設定した過電流基準を超えたか判定します。現在の逆流遮断の判断は、別の検出回路からINPへ伝える構成です。
      | 17番 GND：ICの基準電位と放熱用の接続
      | パッケージ底面にある露出パッドです。横に出ている16本の端子とは別に、底面が17番になっています。
      | 現回路では共通GNDへ接続します。入力信号や分圧回路、TIMERなどの基準になるとともに、基板へ熱を逃がします。ゲート駆動の浮動基準であるTSとは分けて接続します。
      | ゲート駆動・検出端子は仕様書p.10、14、実際の端子配置と底面パッドは仕様書p.3で確認できます。
      | 用語と記号          ; IC：Integrated Circuit（集積回路）。GND：Ground（共通の基準電位・電流帰路）。MCU：Microcontroller Unit（マイコン）。High/Low：デジタル信号の高/低レベル。UV：Under Voltage（低電圧）、OV：Over Voltage（過電圧）、OC：Over Current（過電流）。SOA：Safe Operating Area（安全動作領域）。末尾NはLowで有効になる信号を表す。
      mask Display: text(0.5,0.52,'LTC7000ARMSE','horizontalAlignment','center','texmode','off');text(0.5,0.43,'端子接続図 / 試験モデル対応','horizontalAlignment','center');port_label('lconn',1,'1 RUN');port_label('lconn',2,'2 VIN');port_label('lconn',3,'3 VCC');port_label('lconn',4,'4 VCCUV');port_label('lconn',5,'5 FAULT_N');port_label('lconn',6,'6 TIMER');port_label('lconn',7,'7 INP');port_label('lconn',8,'8 OVLO');port_label('rconn',1,'16 SNS+');port_label('rconn',2,'15 SNS-');port_label('rconn',3,'14 BST');port_label('rconn',4,'13 TS');port_label('rconn',5,'12 TGUP');port_label('rconn',6,'11 TGDN');port_label('rconn',7,'10 IMON');port_label('rconn',8,'9 ISET');port_label('lconn',9,'17 EP GND');
  PV_U3 : Subsystem  Description=|
      | この回路での名前    ; PV_U3
      | 部品名              ; TLV3201AIDBVR
      | この回路での役割    ; 逆流が設定値を超えたか比較し、プログラムを待たず停止条件を作る。
      | ここでの動き        ; IPV_OUTとしきい値V_REVを比べ、逆流が設定量を超えるとREV_OKをLowへ下げる。ADC用R25/C23の手前から読むため、遅いADCフィルタやMicroPythonの読み取り待ちに依存せず停止要求を作る。
      | 読み取りの注意      ; 公称V_REVは約1.225Vで、U2の公称特性なら逆流約−0.5Aに相当する。これは厳密な保証値ではなく、比較器オフセット・ヒステリシス・抵抗公差・測定アンプ誤差で判定幅が生じる。実際のピーク逆流は判定しきい値そのものではなく、検出とゲート放電の遅れにも依存する。
      | 端子と接続          ; 1 OUT → REV_OK、2 GND → GND、3 IN+ → IPV_OUT、5 VCC → P3V3、4 IN- → V_REV
      | パッケージと視点    ; DBV5 SOT-23。メーカー上面図の物理番号順。LTC7000Aの17番露出パッドは実物では裏面、図面では左下へ引き出す。
      | この図の範囲        ; この図面は実部品の端子と接続を示す。保存実行モジュール SHA256=f40bf5e1ef20bc97d0d4775a6ac457f3c30378c5fe9d07d29ab7bde4d975da32 の数値計算用ICコアを図面コピーから除去してある。実行用のICはメーカーのトランジスタモデルではなく、限定範囲の近似動作モデル。試験の合否と条件は C:\Users\hosik\OneDrive\ドキュメント\ChatGPT\oosem\evaluation\pv_protection_integration_20261023_r01\runtime\observations\standard_final_r04_aggregate\aggregate.json を参照する。
      | ソフトウェア確認    ; 試験で与えた指令・境界条件と、RP2040上で動くMicroPythonプログラムの実行確認は別。今回の記述は実ファームウェアの動作試験を実施したという意味ではない。
      | メーカー根拠        ; https://www.ti.com/lit/ds/symlink/tlv3201.pdf
      | 用語と記号          ; IC：Integrated Circuit（集積回路）。GND：Ground（共通の基準電位・電流帰路）。MCU：Microcontroller Unit（マイコン）。High/Low：デジタル信号の高/低レベル。UV：Under Voltage（低電圧）、OV：Over Voltage（過電圧）、OC：Over Current（過電流）。SOA：Safe Operating Area（安全動作領域）。末尾NはLowで有効になる信号を表す。
      mask Display: text(0.5,0.52,'TLV3201AIDBVR','horizontalAlignment','center','texmode','off');text(0.5,0.43,'端子接続図 / 試験モデル対応','horizontalAlignment','center');port_label('lconn',1,'1 OUT');port_label('lconn',2,'2 GND');port_label('lconn',3,'3 IN+');port_label('rconn',1,'5 VCC');port_label('rconn',2,'4 IN-');
  PV_U4 : Subsystem  Description=|
      | この回路での名前    ; PV_U4
      | 部品名              ; SN74LVC1G11DBVR
      | この回路での役割    ; 逆流なし・アナログ系正常・マイコン許可の3条件をまとめる。
      | ここでの動き        ; REV_OK（逆流停止条件なし）、ANALOG_OK（3.3Vと2.5Vの監視成立）、MCU_RUN（マイコンの通電許可）の3入力をANDでまとめる。1つでもLowならALLOW_CLEAR_NをLowにしてPV_U5を非同期クリアする。ANALOG_OKは同じ保護回路内のPV_U6から生成する。
      | 読み取りの注意      ; 3条件がHighに戻ることは、停止保持を解除できる準備が整ったことを意味する。これだけではMOSFETを自動再投入しない。ANDは全条件成立時だけHighになる論理。
      | 端子と接続          ; 1 A → REV_OK、2 GND → GND、3 B → ANALOG_OK、6 C → MCU_RUN、5 VCC → P3V3、4 Y → ALLOW_CLEAR_N
      | パッケージと視点    ; DBV6 SOT-23。メーカー上面図の物理番号順。LTC7000Aの17番露出パッドは実物では裏面、図面では左下へ引き出す。
      | この図の範囲        ; この図面は実部品の端子と接続を示す。保存実行モジュール SHA256=f40bf5e1ef20bc97d0d4775a6ac457f3c30378c5fe9d07d29ab7bde4d975da32 の数値計算用ICコアを図面コピーから除去してある。実行用のICはメーカーのトランジスタモデルではなく、限定範囲の近似動作モデル。試験の合否と条件は C:\Users\hosik\OneDrive\ドキュメント\ChatGPT\oosem\evaluation\pv_protection_integration_20261023_r01\runtime\observations\standard_final_r04_aggregate\aggregate.json を参照する。
      | ソフトウェア確認    ; 試験で与えた指令・境界条件と、RP2040上で動くMicroPythonプログラムの実行確認は別。今回の記述は実ファームウェアの動作試験を実施したという意味ではない。
      | メーカー根拠        ; https://www.ti.com/lit/ds/symlink/sn74lvc1g11.pdf
      | 用語と記号          ; IC：Integrated Circuit（集積回路）。GND：Ground（共通の基準電位・電流帰路）。MCU：Microcontroller Unit（マイコン）。High/Low：デジタル信号の高/低レベル。UV：Under Voltage（低電圧）、OV：Over Voltage（過電圧）、OC：Over Current（過電流）。SOA：Safe Operating Area（安全動作領域）。末尾NはLowで有効になる信号を表す。
      mask Display: text(0.5,0.52,'SN74LVC1G11DBVR','horizontalAlignment','center','texmode','off');text(0.5,0.43,'端子接続図 / 試験モデル対応','horizontalAlignment','center');port_label('lconn',1,'1 A');port_label('lconn',2,'2 GND');port_label('lconn',3,'3 B');port_label('rconn',1,'6 C');port_label('rconn',2,'5 VCC');port_label('rconn',3,'4 Y');
  PV_U5 : Subsystem  Description=|
      | この回路での名前    ; PV_U5
      | 部品名              ; SN74LVC1G74DCTR
      | この回路での役割    ; 逆流などで一度停止した状態を保持し、電流ゼロに戻っただけでは再通電させない。
      | ここでの動き        ; CLR_NがLowならQ=PV_ALLOWをLowへ非同期クリアして停止状態を保持する。Dは3.3Vへ固定、PRE_NもHighで通常は無効。3条件が正常に戻ってもQは自動でHighにならず、MCU_REARMの立上りを受けて初めてD=Highを取り込む。
      | 読み取りの注意      ; 3番Q_N=PV_STOPPEDは反転した保持状態、5番Q=PV_ALLOWは通電許可。PV_STOPPEDは逆流・電源低下などの原因を区別せず、物理MOSFETが遮断できたことの独立測定でもない。電源投入時のフリップフロップ状態を既知と仮定せず、MCU_RUNをLowにしてクリアを確立してから再許可する。
      | 端子と接続          ; 1 CLK → MCU_REARM、2 D → P3V3、3 Q_N → PV_STOPPED、4 GND → GND、8 VCC → P3V3、7 PRE_N → P3V3、6 CLR_N → ALLOW_CLEAR_N、5 Q → PV_ALLOW
      | パッケージと視点    ; DCT8 SM8。メーカー上面図の物理番号順。LTC7000Aの17番露出パッドは実物では裏面、図面では左下へ引き出す。
      | この図の範囲        ; この図面は実部品の端子と接続を示す。保存実行モジュール SHA256=f40bf5e1ef20bc97d0d4775a6ac457f3c30378c5fe9d07d29ab7bde4d975da32 の数値計算用ICコアを図面コピーから除去してある。実行用のICはメーカーのトランジスタモデルではなく、限定範囲の近似動作モデル。試験の合否と条件は C:\Users\hosik\OneDrive\ドキュメント\ChatGPT\oosem\evaluation\pv_protection_integration_20261023_r01\runtime\observations\standard_final_r04_aggregate\aggregate.json を参照する。
      | ソフトウェア確認    ; 試験で与えた指令・境界条件と、RP2040上で動くMicroPythonプログラムの実行確認は別。今回の記述は実ファームウェアの動作試験を実施したという意味ではない。
      | メーカー根拠        ; https://www.ti.com/lit/gpn/sn74lvc1g74
      | 用語と記号          ; IC：Integrated Circuit（集積回路）。GND：Ground（共通の基準電位・電流帰路）。MCU：Microcontroller Unit（マイコン）。High/Low：デジタル信号の高/低レベル。UV：Under Voltage（低電圧）、OV：Over Voltage（過電圧）、OC：Over Current（過電流）。SOA：Safe Operating Area（安全動作領域）。末尾NはLowで有効になる信号を表す。
      mask Display: text(0.5,0.52,'SN74LVC1G74DCTR','horizontalAlignment','center','texmode','off');text(0.5,0.43,'端子接続図 / 試験モデル対応','horizontalAlignment','center');port_label('lconn',1,'1 CLK');port_label('lconn',2,'2 D');port_label('lconn',3,'3 Q_N');port_label('lconn',4,'4 GND');port_label('rconn',1,'8 VCC');port_label('rconn',2,'7 PRE_N');port_label('rconn',3,'6 CLR_N');port_label('rconn',4,'5 Q');
  PV_U6 : Subsystem  Description=|
      | この回路での名前    ; PV_U6
      | 部品名              ; TPS37042BJOFDDFRQ1
      | この回路での役割    ; 電流判定に使う3.3V電源と2.5V基準電源が使える状態か監視するIC。2系統とも正常のときだけANALOG_OKを許す。
      | ここでの動き        ; VDDは3.3Vから供給する。SENSE1は3.3Vを31.2kΩ/10kΩで、SENSE2は2.5Vを21.3kΩ/10kΩで分圧して監視する。2本のオープンドレインRESETを同じANALOG_OKへつなぎ、10kΩで3.3Vへ引き上げる。どちらか異常ならLowへ引き下げ、両方正常に戻って復帰待ち時間を過ぎたら解放する。
      | 設定の意味          ; 選択型番は調整式の公称0.8V±4%窓、復帰待ち公称10ms。しきい値公差・ヒステリシス・漏れ電流・検出遅延の条件はメーカー資料と試験記録を参照。
      | 起動時の注意        ; 電源が極端に低い間の出力は無条件に保証されない。ANALOG_OKだけに起動時OFFを任せず、MCU_RUN Lowとゲート/入力の受動部品も合わせて評価する。
      | 端子と接続          ; 1 VDD → P3V3、2 SENSE1 → PV_SUP_3V3、3 SENSE2 → PV_SUP_2V5、4 GND → GND、8 RESET1n → ANALOG_OK、7 RESET2n → ANALOG_OK、6 NC6 → NC（未接続）、5 NC5 → NC（未接続）
      | パッケージと視点    ; DDF, SOT-23-8, top view
      | この図の範囲        ; この図面は実部品の端子と接続を示す。保存実行モジュール SHA256=f40bf5e1ef20bc97d0d4775a6ac457f3c30378c5fe9d07d29ab7bde4d975da32 の数値計算用ICコアを図面コピーから除去してある。実行用のICはメーカーのトランジスタモデルではなく、限定範囲の近似動作モデル。試験の合否と条件は C:\Users\hosik\OneDrive\ドキュメント\ChatGPT\oosem\evaluation\pv_protection_integration_20261023_r01\runtime\observations\standard_final_r04_aggregate\aggregate.json を参照する。
      | ソフトウェア確認    ; 試験で与えた指令・境界条件と、RP2040上で動くMicroPythonプログラムの実行確認は別。今回の記述は実ファームウェアの動作試験を実施したという意味ではない。
      | メーカー根拠        ; https://www.ti.com/lit/ds/symlink/tps3704.pdf
      | 用語と記号          ; IC：Integrated Circuit（集積回路）。GND：Ground（共通の基準電位・電流帰路）。MCU：Microcontroller Unit（マイコン）。High/Low：デジタル信号の高/低レベル。UV：Under Voltage（低電圧）、OV：Over Voltage（過電圧）、OC：Over Current（過電流）。SOA：Safe Operating Area（安全動作領域）。末尾NはLowで有効になる信号を表す。 SENSE：監視入力。RESET：リセット出力。オープンドレイン：Lowへの引込みだけを行い、Highは外付け抵抗で作る出力形式。NC：No Connect（接続しない端子）。
      mask Display: disp('TPS37042 / 電源監視');port_label('lconn',1,'1 VDD');port_label('lconn',2,'2 SENSE1');port_label('lconn',3,'3 SENSE2');port_label('lconn',4,'4 GND');port_label('rconn',1,'8 RESET1n');port_label('rconn',2,'7 RESET2n');port_label('rconn',3,'6 NC6');port_label('rconn',4,'5 NC5');
  R27 : Subsystem  Description=|  mask(太陽光充電回路 編集用部品){PartRef=R27, PartMPN=CSS4J-4026R-1L00F, PartValue=1 mOhm / Kelvin, DesignValue=1 mohm, SourceRef=FI_MEAS_FRONTEND/SH_PV}
      | この回路での名前    ; R27
      | 部品名              ; CSS4J-4026R-1L00F
      | この回路での役割    ; パネル電流を測る既存の1 mΩシャント。逆流判定と順方向過電流検出の両方へ渡す。
      | ここでの動き        ; 電力用IP/IMと検出用KP/KMを分ける。候補図ではMOSFET対より上流に置く。このc06図面では元c05のR27を共有して移設し、二重追加しない。
      | モデルの範囲        ; 内部にSimscape標準抵抗を持つ4端子図面。配線寄生・熱は未同定。
      | 略語と記号          ; Kelvin：電力線と検出線を分けて配線電圧降下を混ぜにくくする4端子接続。mΩ：ミリオーム。
      mask prompts: PartRef "物理部品番号"; PartMPN "部品型番"; PartValue "部品値・表示値"; DesignValue "元設計値（記録）"; SourceRef "旧参照名（記録）"
      mask help: 回路図編集用です。端子・配線は実際のSimscape接続ですが、部品内部の動作式は未実装です。値・型番を変更し、配線をドラッグして編集できます。
      mask Display:
      | color('black');
      | plot([0 .30 .30 .35],[0.181818 0.181818 .5 .5]);
      | plot([0 .30 .30],[0.818182 0.818182 .5]);
      | plot([0 .13 .13 .70 .70],[0.5 0.5 .94 .94 .5]);
      | plot([.35 .35 .65 .65 .35],[.35 .65 .65 .35 .35]);
      | plot([.65 .70 .70 1],[.5 .5 0.5 0.5]);
      | text(0,0.261818,'IP','horizontalAlignment','left');
      | text(0,0.898182,'KP','horizontalAlignment','left');
      | text(0,0.58,'KM','horizontalAlignment','left');
      | text(1,0.58,'IM','horizontalAlignment','right');
  U2 : Subsystem  Description=|
      | この回路での名前    ; U2
      | 部品名              ; INA241A3IDDFR
      | この回路での役割    ; 既存のパネル電流測定ICを共有し、逆流の有無を低電圧信号で判定できるようにする。
      | ここでの動き        ; 既存のR27とこの測定ICを共有する。PVから充電回路へ流れる電流を正とし、公称出力は1.25V+0.05V/A×電流。REF1=2.5V、REF2=GND。出力IPV_OUTは逆流比較器へ直接渡し、別枝のR25/C23を通してADCへ渡す。
      | 読み取りの注意      ; 4番NC_RESERVEDは名称にNCを含むがメーカー指定に従いGNDへ接続する。追加の2個目の電流測定ICではない。入力コモンモード急変時の保持動作、オフセット、帯域、スルーの全特性を図面が再現する意味ではない。
      | 端子と接続          ; 1 IN- → PV_SENSED、2 GND → GND、3 REF2 → GND、4 NC_RESERVED → GND、8 IN+ → PV_IN、7 REF1 → VREF2V5、6 VS → P3V3、5 OUT → IPV_OUT
      | パッケージと視点    ; DDF8 SOT-23。メーカー上面図の物理番号順。LTC7000Aの17番露出パッドは実物では裏面、図面では左下へ引き出す。
      | この図の範囲        ; この図面は実部品の端子と接続を示す。保存実行モジュール SHA256=f40bf5e1ef20bc97d0d4775a6ac457f3c30378c5fe9d07d29ab7bde4d975da32 の数値計算用ICコアを図面コピーから除去してある。実行用のICはメーカーのトランジスタモデルではなく、限定範囲の近似動作モデル。試験の合否と条件は C:\Users\hosik\OneDrive\ドキュメント\ChatGPT\oosem\evaluation\pv_protection_integration_20261023_r01\runtime\observations\standard_final_r04_aggregate\aggregate.json を参照する。
      | ソフトウェア確認    ; 試験で与えた指令・境界条件と、RP2040上で動くMicroPythonプログラムの実行確認は別。今回の記述は実ファームウェアの動作試験を実施したという意味ではない。
      | メーカー根拠        ; https://www.ti.com/lit/ds/symlink/ina241a.pdf
      | 用語と記号          ; IC：Integrated Circuit（集積回路）。GND：Ground（共通の基準電位・電流帰路）。MCU：Microcontroller Unit（マイコン）。High/Low：デジタル信号の高/低レベル。UV：Under Voltage（低電圧）、OV：Over Voltage（過電圧）、OC：Over Current（過電流）。SOA：Safe Operating Area（安全動作領域）。末尾NはLowで有効になる信号を表す。
      mask Display: text(0.5,0.52,'INA241A3IDDFR','horizontalAlignment','center','texmode','off');text(0.5,0.43,'端子接続図 / 試験モデル対応','horizontalAlignment','center');port_label('lconn',1,'1 IN-');port_label('lconn',2,'2 GND');port_label('lconn',3,'3 REF2');port_label('lconn',4,'4 NC_RESERVED');port_label('rconn',1,'8 IN+');port_label('rconn',2,'7 REF1');port_label('rconn',3,'6 VS');port_label('rconn',4,'5 OUT');
  IF_PV_IN : PMIOPort  Description=|  Side=Left  ConnectionType=Connection: foundation.electrical.electrical
      | 接続名              ; PV_IN
      | この接続の役割      ; パネル/L2側、シャントより上流の正極
      | 外部への接続        ; 候補サブサーキットの接続口。外部回路・生成元はこのモデルに含まない。
  IF_PV_OUT : PMIOPort  Description=|  Port=2  Side=Right  ConnectionType=Connection: foundation.electrical.electrical
      | 接続名              ; PV_OUT
      | この接続の役割      ; 充電回路入力コンデンサ側正極
      | 外部への接続        ; 候補サブサーキットの接続口。外部回路・生成元はこのモデルに含まない。
  IF_GND : PMIOPort  Description=|  Port=3  Side=Left  ConnectionType=Connection: foundation.electrical.electrical
      | 接続名              ; GND
      | この接続の役割      ; 主回路と共通の基準電位
      | 外部への接続        ; 候補サブサーキットの接続口。外部回路・生成元はこのモデルに含まない。
  IF_P3V3 : PMIOPort  Description=|  Port=4  Side=Left  ConnectionType=Connection: foundation.electrical.electrical
      | 接続名              ; P3V3
      | この接続の役割      ; 既存3.3V電源。電源立上り・消失条件は要検証
      | 外部への接続        ; 候補サブサーキットの接続口。外部回路・生成元はこのモデルに含まない。
  IF_VREF2V5 : PMIOPort  Description=|  Port=5  Side=Left  ConnectionType=Connection: foundation.electrical.electrical
      | 接続名              ; VREF2V5
      | この接続の役割      ; 既存2.5V基準電源。ここでは新しい基準ICを追加しない
      | 外部への接続        ; 候補サブサーキットの接続口。外部回路・生成元はこのモデルに含まない。
  IF_MCU_RUN : PMIOPort  Description=|  Port=6  Side=Left  ConnectionType=Connection: foundation.electrical.electrical
      | 接続名              ; MCU_RUN
      | この接続の役割      ; マイコン運転許可。起動時Low、異常/停止でLow
      | 外部への接続        ; 候補サブサーキットの接続口。外部回路・生成元はこのモデルに含まない。
  IF_MCU_REARM : PMIOPort  Description=|  Port=7  Side=Left  ConnectionType=Connection: foundation.electrical.electrical
      | 接続名              ; MCU_REARM
      | この接続の役割      ; 条件がそろった後の手動再許可立上りパルス
      | 外部への接続        ; 候補サブサーキットの接続口。外部回路・生成元はこのモデルに含まない。
  IF_IPV_OUT : PMIOPort  Description=|  Port=8  Side=Right  ConnectionType=Connection: foundation.electrical.electrical
      | 接続名              ; IPV_OUT
      | この接続の役割      ; 既存測定系のフィルタ前出力。ADC側へも分岐可能
      | 外部への接続        ; 候補サブサーキットの接続口。外部回路・生成元はこのモデルに含まない。
  IF_OC_FAULT_N : PMIOPort  Description=|  Port=9  Side=Right  ConnectionType=Connection: foundation.electrical.electrical
      | 接続名              ; OC_FAULT_N
      | この接続の役割      ; LTC7000AのFAULT出力。逆流発生の専用通知ではない
      | 外部への接続        ; 候補サブサーキットの接続口。外部回路・生成元はこのモデルに含まない。
  IF_PV_STOPPED : PMIOPort  Description=|  Port=10  Side=Right  ConnectionType=Connection: foundation.electrical.electrical
      | 接続名              ; PV_STOPPED
      | この接続の役割      ; 停止ラッチの反転出力。停止原因や実MOSFET状態を直接保証しない
      | 外部への接続        ; 候補サブサーキットの接続口。外部回路・生成元はこのモデルに含まない。
  connections:
  PV_C_SUP/RConn1 -- GND_01/LConn1
  PV_D_NEG/LConn1 -- GND_02/LConn1
  PV_D_TS/LConn1 -- GND_03/LConn1
  PV_R_SUP26/RConn1 -- GND_04/LConn1
  PV_R_SUP32/RConn1 -- GND_05/LConn1
  PV_U6/LConn4 -- GND_06/LConn1
  IF_GND/RConn1 -- GND_07/LConn1
  PV_CTIME/RConn1 -- GND_08/LConn1
  PV_CVCC/RConn1 -- GND_09/LConn1
  PV_CVIN/RConn1 -- GND_10/LConn1
  PV_C_SLEW/RConn1 -- GND_11/LConn1
  PV_RINP/RConn1 -- GND_12/LConn1
  PV_ROV_L/RConn1 -- GND_13/LConn1
  PV_RTIME/RConn1 -- GND_14/LConn1
  PV_RUV_L/RConn1 -- GND_15/LConn1
  PV_RVCCUV/RConn1 -- GND_16/LConn1
  PV_U1/LConn9 -- GND_17/LConn1
  PV_U1/RConn8 -- GND_18/LConn1
  C22/RConn1 -- GND_19/LConn1
  PV_CREV/RConn1 -- GND_20/LConn1
  PV_C_PV_U3/RConn1 -- GND_21/LConn1
  PV_RREV_L/RConn1 -- GND_22/LConn1
  PV_U3/LConn2 -- GND_23/LConn1
  U2/LConn2 -- GND_24/LConn1
  U2/LConn3 -- GND_25/LConn1
  U2/LConn4 -- GND_26/LConn1
  PV_C_PV_U4/RConn1 -- GND_27/LConn1
  PV_C_PV_U5/RConn1 -- GND_28/LConn1
  PV_RAN/RConn1 -- GND_29/LConn1
  PV_RREARM/RConn1 -- GND_30/LConn1
  PV_RRUN/RConn1 -- GND_31/LConn1
  PV_U4/LConn2 -- GND_32/LConn1
  PV_U5/LConn4 -- GND_33/LConn1
  PV_CVCC/LConn1 -- PV_U1/LConn3 -- PV_D_BOOT/LConn1
  PV_U1/RConn3 -- PV_CBST/LConn1 -- PV_D_BOOT/RConn1
  PV_Q1/LConn1 -- PV_Q2/LConn1 -- PV_D_GS/RConn1 -- PV_RGS/LConn1 -- PV_RG/RConn1 -- PV_U1/RConn6 -- PV_R_SLEW/LConn1
  PV_C_SLEW/LConn1 -- PV_R_SLEW/RConn1
  PV_U1/RConn5 -- PV_RG/LConn1
  PV_Q1/RConn2 -- PV_D_GS/LConn1 -- PV_RGS/RConn1 -- PV_CBST/RConn1 -- PV_U1/RConn4 -- PV_Q2/RConn2 -- PV_D_TS/RConn1
  PV_U1/RConn2 -- PV_RFLT/RConn1
  PV_RUV_H/RConn1 -- PV_RUV_L/LConn1 -- PV_U1/LConn1
  PV_RVCCUV/LConn1 -- PV_U1/LConn4
  PV_RTIME/LConn1 -- PV_CTIME/LConn1 -- PV_U1/LConn6
  PV_RINP/LConn1 -- PV_U5/RConn4 -- PV_U1/LConn7
  PV_ROV_H/RConn1 -- PV_ROV_L/LConn1 -- PV_U1/LConn8
  PV_D_FLY/LConn1 -- L2/RConn1 -- PV_Q1/RConn1 -- PV_D_NEG/RConn1
  IF_PV_OUT/RConn1 -- PV_Q2/RConn1
  PV_R_SUP32/LConn1 -- PV_R_SUP31/RConn1 -- PV_U6/LConn2
  PV_R_SUP26/LConn1 -- PV_R_SUP25/RConn1 -- PV_U6/LConn3
  IF_IPV_OUT/RConn1 -- PV_U3/LConn3 -- U2/RConn4
  PV_U3/RConn2 -- PV_RREV_H/RConn1 -- PV_CREV/LConn1 -- PV_RREV_L/LConn1
  IF_P3V3/RConn1 -- PV_R_SUP31/LConn1 -- PV_C_SUP/LConn1 -- PV_R_SUP_PU/LConn1 -- PV_U4/RConn2 -- PV_C_PV_U4/LConn1 -- PV_U5/LConn2 -- PV_U5/RConn2 -- PV_C_PV_U5/LConn1 -- PV_U5/RConn1 -- PV_U6/LConn1 -- PV_C_PV_U3/LConn1 -- PV_U3/RConn1 -- C22/LConn1 -- U2/RConn3 -- PV_RFLT_PU/LConn1
  PV_D_FLY/RConn1 -- R27/LConn2 -- R27/RConn1 -- Connection Label1/LConn1 -- L2/LConn1
  IF_VREF2V5/RConn1 -- PV_RREV_H/LConn1 -- PV_R_SUP25/LConn1 -- U2/RConn2
  Connection Label5/LConn1 -- PV_CVIN/LConn1 -- PV_U1/LConn2 -- PV_RUV_H/LConn1
  IF_MCU_RUN/RConn1 -- PV_U4/RConn1 -- PV_RRUN/LConn1
  IF_MCU_REARM/RConn1 -- PV_RREARM/LConn1 -- PV_U5/LConn1
  IF_PV_STOPPED/RConn1 -- PV_U5/LConn3
  PV_U3/LConn1 -- PV_U4/LConn1
  PV_U4/LConn3 -- PV_RAN/LConn1 -- PV_U6/RConn1 -- PV_U6/RConn2 -- PV_R_SUP_PU/RConn1
  PV_U4/RConn3 -- PV_U5/RConn3
  PV_RFLT_PU/RConn1 -- PV_U1/LConn5 -- IF_OC_FAULT_N/RConn1
  Connection Label/LConn1 -- R27/LConn3 -- IF_PV_IN/RConn1 -- R27/LConn1
  U2/LConn1 -- Connection Label3/LConn1
  Connection Label4/LConn1 -- PV_RFLT/LConn1
  Connection Label6/LConn1 -- U2/RConn1
  Connection Label2/LConn1 -- PV_ROV_H/LConn1
  Connection Label7/LConn1 -- PV_U1/RConn1
